simulink model "FullFMS_2026_02_25_V0_4_31_R2026a"  (R2026a)
settings: Solver=FixedStepAuto  StopTime=inf  FixedStep=0.01  MaxStep=0.01  RelTol=1e-2
PreLoadFcn:
  | load("BUS_CONFIG.mat")
libraries: opcualib x8
(part 3 of 4)

== stateflow chart FullFMS_2026_02_25_V0_4_31_R2026a/Chart ==
  note: Conveyor
  note: Sorting [60]
  state BRS
    entry:
    StatusBRS_5 = false;   % v0.4.29: zera o fim de ciclo anterior
    state STATE1
      entry:
      StatusBRS_1 = false;
      during:
      % Configuracao da estacao: so este bloco fica ativo se o bit dele estiver ligado
      if Control_60.C_65_BRS_Output
      StatusBRS_1 = true;
      else
      StatusBRS_1 = false;
      end
    state ESTATE2
      entry:
      StatusBRS_2 = false;
      during:
      % Janela de identificacao da peca (T1 = 2s no ladder)
      if Control_50.C_55_PD_Sort
      StatusBRS_2 = true;
      else
      StatusBRS_2 = false;
      end
    state ESTATE3
      entry:
      StatusBRS_3 = false;
      during:
      % Preta: SL1 avanca | Vermelha: SL2 avanca | Prata: ambas recuadas
      if ((Control_60.C_65_ID_1 && ~Control_60.C_65_ID_2) && Sensors_60.O_60_SL1_Fwd) || ...
      ((Control_60.C_65_ID_1 && Control_60.C_65_ID_2) && Sensors_60.O_60_SL2_Fwd) || ...
      ((~Control_60.C_65_ID_1 && Control_60.C_65_ID_2) && Sensors_60.O_60_SL1_Bck && Sensors_60.O_60_SL2_Bck)
      StatusBRS_3 = true;
      else
      StatusBRS_3 = false;
      end
    state ESTATE5
      entry:
      StatusBRS_5 = false;
      during:
      % Pino recuado: ciclo concluido, pronto para a proxima peca
      if ~Actuators_60.F_62_Identify
      StatusBRS_5 = true;
      else
      StatusBRS_5 = false;
      end
    state ESTATE4
      entry:
      % captura no mesmo passo da entrada
      StatusBRS_4 = Actuators_60.F_62_Identify;
      during:
      % Pino de identificacao acionado (LEITURA do CLP - sombra nao comanda)
      % latch (v0.4.31): o pino desliga junto com o Part_Pass, uma vez observado nao volta a false
      if Actuators_60.F_62_Identify
      StatusBRS_4 = true;
      end
    (default) -> BRS.STATE1
    BRS.ESTATE2 -> BRS.ESTATE3 : [(Control_60.C_65_ID_1 == true || Control_60.C_65_ID_2 == true || after(2, sec)) && StatusBRS_2 == true]
    BRS.ESTATE3 -> BRS.ESTATE4 : [StatusBRS_3 == true]
    BRS.ESTATE4 -> BRS.ESTATE5 : [(Sensors_60.O_60_Part_Pass == true || Actuators_60.F_62_Identify == false) && StatusBRS_4 == true]
    BRS.STATE1 -> BRS.ESTATE2 : [Control_50.C_55_PD_Sort == true && StatusBRS_1 == true]
  state Start
    during:
    Control_20.C_24_Request
  note: Testing Station [70]
  note: Distribution Station [80]
  state Identified_Delivery
    state Part_HeightSensor
      entry:
      St_IdDl_3a_8 = false;
      during:
      Actuators_70.F_72_Eject_Part;
      Sensors_70.O_70_Pist_Bck;
      Sensors_70.O_70_SPart_Height
      if Actuators_70.F_72_Eject_Part && ...
      ~Sensors_70.O_70_Pist_Bck && ...
      ~Sensors_70.O_70_SPart_Height
      St_IdDl_3a_8 = true;
      else
      St_IdDl_3a_8 = false;
      end
    state Piston_Back
      entry:
      Status3a_10 = false;
      during:
      Actuators_70.F_72_Eject_Part
      if ~Actuators_70.F_72_Eject_Part
      Status3a_10 = true;
      else
      Status3a_10 = false;
      end
    state Elevator_StartsMovingDown
      entry:
      Status3a_11 = false;
      during:
      Actuators_70.F_72_Elev_Down;
      Actuators_70.F_72_Elev_Up;
      if Actuators_70.F_72_Elev_Down && ...
      ~Actuators_70.F_72_Elev_Up
      Status3a_11 = true;
      else
      Status3a_11 = false;
      end
    state Elevator_MiddleDown
      entry:
      Status3a_12 = false;
      during:
      Sensors_70.O_70_SStation;
      if ~Sensors_70.O_70_SStation
      Status3a_12 = true;
      else
      Status3a_12 = false;
      end
    state Elevator_InductiveDown
      entry:
      St_IdDl_3a_13 = false;
      during:
      Sensors_70.O_70_SInductive;
      if ~Sensors_70.O_70_SInductive
      St_IdDl_3a_13 = true;
      else
      St_IdDl_3a_13 = false;
      end
    state Pushes_Part
      entry:
      Status3a_7 = false;
      during:
      Actuators_70.F_72_Eject_Part;
      Actuators_70.F_72_Air_On;
      Sensors_70.O_70_SPart;
      if Actuators_70.F_72_Eject_Part && ...
      Actuators_70.F_72_Air_On && ...
      ~Sensors_70.O_70_SPart
      Status3a_7 = true;
      else
      Status3a_7 = false;
      end
    state InitialCondition
      entry:
      St_IdDl_3a_1 = false;
      during:
      AS_i_70.A_74_Cart_Full;
      Control_70.C_75_Initialization;
      Control_70.C_72_Profibus;
      Control_70.C_75_Identified;
      Sensors_70.O_70_SPart;
      Sensors_70.O_71_Key_Pos;
      if ~AS_i_70.A_74_Cart_Full && ...
      Control_70.C_75_Initialization && ...
      Control_70.C_72_Profibus && ...
      Control_70.C_75_Identified && ...
      ~Sensors_70.O_70_SPart && ...
      Sensors_70.O_71_Key_Pos
      St_IdDl_3a_1 = true;
      else
      St_IdDl_3a_1 = false;
      end
    state Part_Arrives
      entry:
      Status3a_2 = false;
      during:
      Control_70.C_75_ID_Delivery2;
      Sensors_70.O_70_SInductive;
      Sensors_70.O_70_SPart;
      Sensors_80.O_80_Arm_Mag;
      if Sensors_70.O_70_SPart && ...
      ((Sensors_70.O_70_SInductive && ...
      Control_70.C_75_ID_Delivery2) | ...
      (~Sensors_70.O_70_SInductive && ...
      ~Control_70.C_75_ID_Delivery2)) && ...
      ~Sensors_80.O_80_Arm_Mag
      Status3a_2 = true;
      else
      Status3a_2 =false;
      end
    state Elevator_Up
      entry:
      Status3a_3 = false;
      during:
      Actuators_70.F_72_Elev_Up;
      if Actuators_70.F_72_Elev_Up
      Status3a_3 = true;
      else
      Status3a_3 = false;
      end
    state Elevator_StartsMovingUp
      entry:
      Status3a_4 = false;
      during:
      Sensors_70.O_70_SInductive;
      if ~Sensors_70.O_70_SInductive
      Status3a_4 = true;
      else
      Status3a_4 = false;
      end
    state Elevator_MiddleUp
      entry:
      Status3a_5 = false;
      during:
      Sensors_70.O_70_SStation;
      if ~Sensors_70.O_70_SStation
      Status3a_5 = true;
      else
      Status3a_5 = false;
      end
    state Elevator_High_Identify_Part
      entry:
      Status3a_6 = false;
      during:
      MetalicPart;
      Control_70.C_75_ID_Delivery1;
      Control_70.C_75_ID_Delivery2;
      Sensors_70.O_70_SPart_Height;
      if MetalicPart && ...
      Control_70.C_75_ID_Delivery2 && ...
      ~Control_70.C_75_ID_Delivery1;
      Status3a_6 = true;
      end
      if ~MetalicPart && ...
      Control_70.C_75_ID_Delivery1 && ...
      ((Sensors_70.O_70_SPart_Height && ...
      Control_70.C_75_ID_Delivery2) | ...
      (~Sensors_70.O_70_SPart_Height && ...
      ~Control_70.C_75_ID_Delivery2))
      Status3a_6=true;
      end
    state Elevator_Down
      entry:
      Status3a_14 = false;
      during:
      AS_i_70.A_74_CRoute_Out;
      Actuators_70.F_72_Elev_Down;
      Control_70.C_75_Part_Del;
      if AS_i_70.A_74_CRoute_Out && ...
      ~Actuators_70.F_72_Elev_Down&& ...
      Control_70.C_75_Part_Del
      Status3a_14 = true;
      else
      Status3a_14 = false;
      end
    state Part_ArrivesAtCart
      entry:
      Status3a_9 = false;
      during:
      AS_i_70.A_74_Cart_Full;
      AS_i_70.A_74_Optic;
      Actuators_70.F_72_Air_On;
      Actuators_70.F_73_Led_Extra2
      if AS_i_70.A_74_Optic && ...
      AS_i_70.A_74_Cart_Full && ...
      ~Actuators_70.F_72_Air_On && ...
      Actuators_70.F_73_Led_Extra2;
      Status3a_9 = true;
      else
      Status3a_9 = false;
      end
    state End_Process
      entry:
      Status3a_15 = false;
      during:
      AS_i_70.A_74_CRoute_Out;
      if  ~AS_i_70.A_74_CRoute_Out
      Status3a_15 = true;
      else
      Status3a_15 = false;
      end
    state Metalic_Identify
      entry:
      MetalicPart = false;
      during:
      Sensors_70.O_70_SInductive;
      if Sensors_70.O_70_SInductive
      MetalicPart = true;
      else
      MetalicPart = false;
      end
    (default) -> Identified_Delivery.InitialCondition
    Identified_Delivery.Elevator_StartsMovingDown -> Identified_Delivery.Elevator_MiddleDown : [Status3a_11 == true && ...
        | Sensors_70.O_70_SStation == true]
    Identified_Delivery.Piston_Back -> Identified_Delivery.Elevator_StartsMovingDown : [Status3a_10 == true && ...
        | Sensors_70.O_70_Pist_Bck == true]
    Identified_Delivery.Elevator_MiddleDown -> Identified_Delivery.Elevator_InductiveDown : [Status3a_12 == true && ...
        | Sensors_70.O_70_SInductive == true]
    Identified_Delivery.Part_Arrives -> Identified_Delivery.Elevator_Up : [Status3a_2 == true && ...
        | Sensors_80.O_80_Arm_Mag == true ]
    Identified_Delivery.Elevator_High_Identify_Part -> Identified_Delivery.Pushes_Part : [Status3a_6 == true && ...
        | (Actuators_70.F_72_Eject_Part == true || after(2, sec))]
    Identified_Delivery.Pushes_Part -> Identified_Delivery.Part_HeightSensor : [Status3a_7 == true && ...
        | Sensors_70.O_70_Pist_Bck == false]
    Identified_Delivery.Elevator_Up -> Identified_Delivery.Elevator_StartsMovingUp : [Status3a_3 == true && ...
        | Sensors_70.O_70_SInductive == true ]
    Identified_Delivery.Elevator_InductiveDown -> Identified_Delivery.Elevator_Down : [St_IdDl_3a_13 == true && ...
        | Sensors_70.O_70_Elev_Low == true]
    Identified_Delivery.Part_HeightSensor -> (junction 1354)
    (junction 1354) -> Identified_Delivery.Piston_Back [order 1] : [St_IdDl_3a_8 == true && ...
        | (Sensors_70.O_70_Pist_Bck == true || after(2, sec))]
    Identified_Delivery.Elevator_StartsMovingUp -> Identified_Delivery.Elevator_MiddleUp : [Status3a_4 == true && ...
        | Sensors_70.O_70_SStation == true]
    Identified_Delivery.Elevator_MiddleUp -> Identified_Delivery.Elevator_High_Identify_Part : [Status3a_5 == true && ...
        | Sensors_70.O_70_Elev_High == true]
    Identified_Delivery.InitialCondition -> (junction 1348) : [St_IdDl_3a_1 == true && ...
        | Sensors_70.O_70_SPart == true]
    (junction 1348) -> Identified_Delivery.Part_Arrives [order 1]
    (junction 1354) -> (junction 1356) [order 2] : [St_IdDl_3a_8 == true && ...
        | AS_i_70.A_74_Optic == true]
    (junction 1348) -> (junction 1350) [order 2]
    Identified_Delivery.Elevator_Down -> Identified_Delivery.End_Process : [Sensors_70.O_70_Elev_Low == true && Control_70.C_75_Part_Del == true]
    (junction 1356) -> Identified_Delivery.Part_ArrivesAtCart
    (junction 1350) -> Identified_Delivery.Metalic_Identify
  state Distribution_Single
    state PistonStartsMoveBackward
      entry:
      St_DSg0_2a_7 = false;
      during:
      Sensors_80.O_80_Pist_Fwd;
      if ~Sensors_80.O_80_Pist_Fwd
      St_DSg0_2a_7 = true;
      else
      St_DSg0_2a_7 = false;
      end
    state PartFed
      entry:
      St_DSg0_2a_6 = false;
      during:
      Actuators_80.F_82_Pist_Adv;
      if ~Actuators_80.F_82_Pist_Adv
      St_DSg0_2a_6 = true;
      else
      St_DSg0_2a_6 = false;
      end
    state ArmToMagazine
      entry:
      St_DSg0_2a_8 = false;
      during:
      Actuators_80.F_82_Arm_2_Mag;
      if Actuators_80.F_82_Arm_2_Mag
      St_DSg0_2a_8 = true;
      else
      St_DSg0_2a_8 = false;
      end
    state ArmCloseDeliver1
      entry:
      St_DSg0_2a_9 = false;
      during:
      Sensors_70.O_70_SStation;
      if Sensors_70.O_70_SStation
      St_DSg0_2a_9 = true;
      else
      St_DSg0_2a_9 = false;
      end
    state ArmArrives_PicksPart
      entry:
      St_DSg0_2a_10 = false;
      during:
      Actuators_80.F_82_Suction_On;
      Actuators_80.F_82_Arm_2_Mag;
      if Actuators_80.F_82_Suction_On && ...
      ~Actuators_80.F_82_Arm_2_Mag
      St_DSg0_2a_10 = true;
      else
      St_DSg0_2a_10 = false;
      end
    state ArmToDelivery1
      entry:
      St_DSg0_2a_11 = false;
      during:
      Actuators_80.F_82_Arm_2_Del
      if Actuators_80.F_82_Arm_2_Del
      St_DSg0_2a_11 = true;
      else
      St_DSg0_2a_11 = false;
      end
    state ArmCloseDelivery2
      entry:
      St_DSg0_2a_12 = false;
      during:
      Sensors_70.O_70_SStation;
      if Sensors_70.O_70_SStation
      St_DSg0_2a_12 = true;
      else
      St_DSg0_2a_12 = false;
      end
    state ArmArrives_DeliversPart
      entry:
      St_DSg0_2a_13 = false;
      during:
      Actuators_80.F_82_Suction_On;
      Actuators_80.F_82_Suction_Off;
      Actuators_80.F_82_Arm_2_Del;
      if ~Actuators_80.F_82_Suction_On && ...
      Actuators_80.F_82_Suction_Off && ...
      ~Actuators_80.F_82_Arm_2_Del
      St_DSg0_2a_13 = true;
      else
      St_DSg0_2a_13 = false;
      end
    state ArmToMagazine1
      entry:
      St_DSg0_2a_14 = false;
      during:
      Actuators_80.F_82_Suction_Off;
      Actuators_80.F_82_Arm_2_Mag;
      Actuators_80.F_83_Led_Extra1;
      Control_80.C_85_Part_Del;
      if ~Actuators_80.F_82_Suction_Off && ...
      Actuators_80.F_82_Arm_2_Mag && ...
      Actuators_80.F_83_Led_Extra1 && ...
      Control_80.C_85_Part_Del
      St_DSg0_2a_14 = true;
      else
      St_DSg0_2a_14 = false;
      end
    state ArmCloseDeliver3
      entry:
      St_DSg0_2a_15 = false;
      during:
      Sensors_70.O_70_SStation;
      if Sensors_70.O_70_SStation
      St_DSg0_2a_15 = true;
      else
      St_DSg0_2a_15 = false;
      end
    state ArmArrives_Finish
      entry:
      St_DSg0_2a_16 = false;
      during:
      Actuators_80.F_82_Arm_2_Mag;
      if ~Actuators_80.F_82_Arm_2_Mag
      St_DSg0_2a_16 = true;
      else
      St_DSg0_2a_16 = false;
      end
    state InitialCondition
      entry:
      St_DSg0_2a_1 = false;
      during:
      Control_80.C_85_Initialization;
      Control_80.C_86_Mag_Parts;
      Control_80.C_82_Profibus;
      Control_80.C_85_Single;
      Sensors_80.O_80_Arm_Mag;
      Sensors_80.O_81_Key_Pos;
      if Control_80.C_85_Initialization&& ...
      Control_80.C_86_Mag_Parts ~= 0 && ...
      Control_80.C_82_Profibus && ...
      Control_80.C_85_Single && ...
      Sensors_80.O_80_Arm_Mag && ...
      Sensors_80.O_81_Key_Pos
      St_DSg0_2a_1 = true;
      else
      St_DSg0_2a_1 = false;
      end
    state ArmToDelivery
      entry:
      St_DSg0_2a_2 = false;
      during:
      Actuators_80.F_82_Arm_2_Del;
      if Actuators_80.F_82_Arm_2_Del
      St_DSg0_2a_2 = true;
      else
      St_DSg0_2a_2 = false;
      end
    state ArmCloseDelivery
      entry:
      St_DSg0_2a_3 = false;
      during:
      Sensors_70.O_70_SStation;
      if Sensors_70.O_70_SStation
      St_DSg0_2a_3 = true;
      else
      St_DSg0_2a_3 = false;
      end
    state ArmArrives_FeedsPart
      entry:
      St_DSg0_2a_4 = false;
      during:
      Actuators_80.F_82_Pist_Adv;
      Actuators_80.F_82_Arm_2_Del;
      if Actuators_80.F_82_Pist_Adv && ...
      ~Actuators_80.F_82_Arm_2_Del
      St_DSg0_2a_4 = true;
      else
      St_DSg0_2a_4 = false;
      end
    state PistonStartsMoveForward
      entry:
      St_DSg0_2a_5 = false;
      during:
      Sensors_80.O_80_Pist_Bck;
      if ~Sensors_80.O_80_Pist_Bck
      St_DSg0_2a_5 = true;
      else
      St_DSg0_2a_5 = false;
      end
    state T1
      during:
      Control_80.C_85_Part_Del
      Actuators_80.F_83_Led_Extra1
    (default) -> Distribution_Single.InitialCondition
    Distribution_Single.ArmToMagazine1 -> (junction 650)
    (junction 650) -> Distribution_Single.ArmCloseDeliver3 [order 1] : [Sensors_80.O_80_Arm_Del == false &&...
        |  St_DSg0_2a_14 == true]
    Distribution_Single.ArmToDelivery -> Distribution_Single.ArmCloseDelivery : [Sensors_80.O_80_Arm_Mag == false &&...
        |  St_DSg0_2a_2 == true]
    Distribution_Single.ArmCloseDelivery -> Distribution_Single.ArmArrives_FeedsPart : [Sensors_80.O_80_Arm_Del == true && ...
        | St_DSg0_2a_3 == true]
    Distribution_Single.ArmArrives_DeliversPart -> Distribution_Single.ArmToMagazine1 : [Sensors_80.O_80_Part_Stuck == false && ...
        | St_DSg0_2a_13 == true]
    Distribution_Single.ArmCloseDelivery2 -> Distribution_Single.ArmArrives_DeliversPart : [Sensors_80.O_80_Arm_Del == true && ...
        | St_DSg0_2a_12 == true]
    Distribution_Single.ArmArrives_FeedsPart -> Distribution_Single.PistonStartsMoveForward : [St_DSg0_2a_4 == true]
    Distribution_Single.PistonStartsMoveBackward -> Distribution_Single.ArmToMagazine : [Sensors_80.O_80_Pist_Bck == true && ...
        | St_DSg0_2a_7 == true]
    Distribution_Single.ArmCloseDeliver1 -> Distribution_Single.ArmArrives_PicksPart : [Sensors_80.O_80_Arm_Mag == true && ...
        | St_DSg0_2a_9 == true]
    Distribution_Single.PartFed -> Distribution_Single.PistonStartsMoveBackward : [St_DSg0_2a_6 == true]
    Distribution_Single.ArmToMagazine -> Distribution_Single.ArmCloseDeliver1 : [Sensors_80.O_80_Arm_Del == false &&...
        | St_DSg0_2a_8 == true]
    Distribution_Single.InitialCondition -> Distribution_Single.ArmToDelivery : [Sensors_80.O_81_Start == true | ...
        | Control_80.C_85_Start == true | ...
        | Control_70.C_75_RQ_Wrong == true | ...
        | (AS_i_70.A_74_CRoute_In80 == true && Sensors_80.O_81_Key_Pos == true) ]
    Distribution_Single.ArmCloseDeliver3 -> Distribution_Single.ArmArrives_Finish : [Sensors_80.O_80_Arm_Mag == true && ...
        | St_DSg0_2a_15 == true]
    Distribution_Single.ArmToDelivery1 -> Distribution_Single.ArmCloseDelivery2 : [Sensors_80.O_80_Arm_Mag == false &&...
        | St_DSg0_2a_11 == true]
    Distribution_Single.PistonStartsMoveForward -> Distribution_Single.PartFed : [Sensors_80.O_80_Pist_Fwd == true && ...
        | St_DSg0_2a_5 == true]
    Distribution_Single.ArmArrives_PicksPart -> Distribution_Single.ArmToDelivery1 : [Sensors_80.O_80_Part_Stuck == true && ...
        | St_DSg0_2a_10 == true]
    (junction 650) -> (junction 1222) [order 2] : after(4,sec)
    (junction 1222) -> Distribution_Single.T1
  state BSR
    entry:
    StatusBSR_5 = false;   % v0.4.29: zera o fim de ciclo anterior
    state STATE1
      entry:
      StatusBSR_1 = false;
      during:
      % Configuracao da estacao: so este bloco fica ativo se o bit dele estiver ligado
      if Control_60.C_65_BSR_Output
      StatusBSR_1 = true;
      else
      StatusBSR_1 = false;
      end
    state ESTATE2
      entry:
      StatusBSR_2 = false;
      during:
      % Janela de identificacao da peca (T1 = 2s no ladder)
      if Control_50.C_55_PD_Sort
      StatusBSR_2 = true;
      else
      StatusBSR_2 = false;
      end
    state ESTATE3
      entry:
      StatusBSR_3 = false;
      during:
      % Preta: SL1 avanca | Prata: SL2 avanca | Vermelha: ambas recuadas
      if ((Control_60.C_65_ID_1 && ~Control_60.C_65_ID_2) && Sensors_60.O_60_SL1_Fwd) || ...
      ((~Control_60.C_65_ID_1 && Control_60.C_65_ID_2) && Sensors_60.O_60_SL2_Fwd) || ...
      ((Control_60.C_65_ID_1 && Control_60.C_65_ID_2) && Sensors_60.O_60_SL1_Bck && Sensors_60.O_60_SL2_Bck)
      StatusBSR_3 = true;
      else
      StatusBSR_3 = false;
      end
    state ESTATE4
      entry:
      % captura no mesmo passo da entrada
      StatusBSR_4 = Actuators_60.F_62_Identify;
      during:
      % Pino de identificacao acionado (LEITURA do CLP - sombra nao comanda)
      % latch (v0.4.31): o pino desliga junto com o Part_Pass, uma vez observado nao volta a false
      if Actuators_60.F_62_Identify
      StatusBSR_4 = true;
      end
    state ESTATE5
      entry:
      StatusBSR_5 = false;
      during:
      % Pino recuado: ciclo concluido, pronto para a proxima peca
      if ~Actuators_60.F_62_Identify
      StatusBSR_5 = true;
      else
      StatusBSR_5 = false;
      end
    (default) -> BSR.STATE1
    BSR.ESTATE3 -> BSR.ESTATE4 : [StatusBSR_3 == true]
    BSR.ESTATE2 -> BSR.ESTATE3 : [(Control_60.C_65_ID_1 == true || Control_60.C_65_ID_2 == true || after(2, sec)) && StatusBSR_2 == true]
    BSR.STATE1 -> BSR.ESTATE2 : [Control_50.C_55_PD_Sort == true && StatusBSR_1 == true]
    BSR.ESTATE4 -> BSR.ESTATE5 : [(Sensors_60.O_60_Part_Pass == true || Actuators_60.F_62_Identify == false) && StatusBSR_4 == true]
  note: Handling 1 [50]
  state Distribution_Continuous
    state InitialCondition
      entry:
      St_DCt0_2b_1 = false;
      during:
      Control_80.C_85_Initialization;
      Control_80.C_86_Mag_Parts;
      Control_80.C_82_Profibus;
      Control_80.C_85_Continuous;
      Sensors_80.O_80_Arm_Mag;
      Sensors_80.O_81_Key_Pos;
      if Control_80.C_85_Initialization&& ...
      Control_80.C_86_Mag_Parts ~= 0 && ...
      Control_80.C_82_Profibus && ...
      Control_80.C_85_Continuous && ...
      Sensors_80.O_80_Arm_Mag && ...
      Sensors_80.O_81_Key_Pos
      St_DCt0_2b_1 = true;
      else
      St_DCt0_2b_1 = false;
      end
    state ArmToDelivery
      entry:
      St_DCt0_2b_2 = false;
      during:
      Actuators_80.F_82_Arm_2_Del
      if Actuators_80.F_82_Arm_2_Del
      St_DCt0_2b_2 = true;
      else
      St_DCt0_2b_2 = false;
      end
    state ArmCloseDelivery
      entry:
      St_DCt0_2b_3 = false;
      during:
      Sensors_70.O_70_SStation;
      if Sensors_70.O_70_SStation
      St_DCt0_2b_3 = true;
      else
      St_DCt0_2b_3 = false;
      end
    state ArmArrives_FeedsPart
      entry:
      St_DCt0_2b_4 = false;
      during:
      Actuators_80.F_82_Pist_Adv;
      Actuators_80.F_82_Arm_2_Del;
      if Actuators_80.F_82_Pist_Adv && ...
      ~Actuators_80.F_82_Arm_2_Del
      St_DCt0_2b_4 = true;
      else
      St_DCt0_2b_4 = false;
      end
    state PistonStartsMoveForward
      entry:
      St_DCt0_2b_5 = false;
      during:
      Sensors_80.O_80_Pist_Bck;
      if ~Sensors_80.O_80_Pist_Bck
      St_DCt0_2b_5 = true;
      else
      St_DCt0_2b_5 = false;
      end
    state PartFed
      entry:
      St_DCt0_2b_6 = false;
      during:
      Actuators_80.F_82_Pist_Adv;
      if ~Actuators_80.F_82_Pist_Adv
      St_DCt0_2b_6 = true;
      else
      St_DCt0_2b_6 = false;
      end
    state PistonStartsMoveBackward
      entry:
      St_DCt0_2b_7 = false;
      during:
      Sensors_80.O_80_Pist_Fwd;
      if ~Sensors_80.O_80_Pist_Fwd
      St_DCt0_2b_7 = true;
      else
      St_DCt0_2b_7 = false;
      end
    state ArmToMagazine
      entry:
      St_DCt0_2b_8 = false;
      during:
      Actuators_80.F_82_Arm_2_Mag;
      if Actuators_80.F_82_Arm_2_Mag
      St_DCt0_2b_8 = true;
      else
      St_DCt0_2b_8 = false;
      end
    state ArmCloseDeliver1
      entry:
      St_DCt0_2b_9 = false;
      during:
      Sensors_70.O_70_SStation;
      if Sensors_70.O_70_SStation
      St_DCt0_2b_9 = true;
      else
      St_DCt0_2b_9 = false;
      end
    state ArmArrives_PicksPart
      entry:
      St_DCt0_2b_10 = false;
      during:
      Actuators_80.F_82_Suction_On;
      Actuators_80.F_82_Arm_2_Mag;
      if Actuators_80.F_82_Suction_On && ...
      ~Actuators_80.F_82_Arm_2_Mag
      St_DCt0_2b_10 = true;
      else
      St_DCt0_2b_10 = false;
      end
    state ArmToDelivery1
      entry:
      St_DCt0_2b_11 = false;
      during:
      Actuators_80.F_82_Arm_2_Del
      if Actuators_80.F_82_Arm_2_Del
      St_DCt0_2b_11 = true;
      else
      St_DCt0_2b_11 = false;
      end
    state ArmCloseDelivery2
      entry:
      St_DCt0_2b_12 = false;
      during:
      Sensors_70.O_70_SStation;
      if Sensors_70.O_70_SStation
      St_DCt0_2b_12 = true;
      else
      St_DCt0_2b_12 = false;
      end
    state ArmArrives_DeliversPart
      entry:
      St_DCt0_2b_13 = false;
      during:
      Actuators_80.F_82_Suction_On;
      Actuators_80.F_82_Suction_Off;
      Actuators_80.F_82_Arm_2_Del;
      if ~Actuators_80.F_82_Suction_On && ...
      Actuators_80.F_82_Suction_Off && ...
      ~Actuators_80.F_82_Arm_2_Del
      St_DCt0_2b_13 = true;
      else
      St_DCt0_2b_13 = false;
      end
    state PartDel_CheckLoop
      entry:
      LoopDistCont = false;
      during:
      Control_80.C_85_Part_Del
      Sensors_80.O_80_Mag_Empty
      if Control_80.C_85_Part_Del && ...
      ~Sensors_80.O_80_Mag_Empty
      LoopDistCont = true;
      else
      LoopDistCont = false;
      end
    state ArmToMagazine1
      entry:
      St_DCt0_2b_14 = false;
      during:
      Actuators_80.F_82_Suction_Off;
      Actuators_80.F_82_Arm_2_Mag;
      Actuators_80.F_83_Led_Extra1;
      Control_80.C_85_Part_Del;
      if ~Actuators_80.F_82_Suction_Off && ...
      Actuators_80.F_82_Arm_2_Mag && ...
      Actuators_80.F_83_Led_Extra1 && ...
      Control_80.C_85_Part_Del
      St_DCt0_2b_14 = true;
      else
      St_DCt0_2b_14 = false;
      end
    state ArmCloseDeliver3
      entry:
      St_DCt0_2b_15 = false;
      during:
      Sensors_70.O_70_SStation;
      if Sensors_70.O_70_SStation
      St_DCt0_2b_15 = true;
      else
      St_DCt0_2b_15 = false;
      end
    state ArmArrives_Finish
      entry:
      St_DCt0_2b_16 = false;
      during:
      Actuators_80.F_82_Arm_2_Mag;
      if ~Actuators_80.F_82_Arm_2_Mag
      St_DCt0_2b_16 = true;
      else
      St_DCt0_2b_16 = false;
      end
    state T1
      during:
      Control_80.C_85_Part_Del
      Actuators_80.F_83_Led_Extra1
    Distribution_Continuous.ArmArrives_PicksPart -> Distribution_Continuous.ArmToDelivery1 : [Sensors_80.O_80_Part_Stuck == true && ...
        | St_DCt0_2b_10 == true]
    Distribution_Continuous.ArmArrives_DeliversPart -> Distribution_Continuous.PartDel_CheckLoop : [Sensors_80.O_80_Part_Stuck == false && ...
        | St_DCt0_2b_13 == true]
    Distribution_Continuous.ArmCloseDelivery -> Distribution_Continuous.ArmArrives_FeedsPart : [Sensors_80.O_80_Arm_Del == true && ...
        | St_DCt0_2b_3 == true]
    Distribution_Continuous.ArmArrives_FeedsPart -> Distribution_Continuous.PistonStartsMoveForward : [St_DCt0_2b_4 == true]
    (default) -> Distribution_Continuous.InitialCondition
    Distribution_Continuous.PartFed -> Distribution_Continuous.PistonStartsMoveBackward : [St_DCt0_2b_6 == true]
    Distribution_Continuous.PistonStartsMoveForward -> Distribution_Continuous.PartFed : [Sensors_80.O_80_Pist_Fwd == true && ...
        | St_DCt0_2b_5 == true]
    Distribution_Continuous.ArmToDelivery -> Distribution_Continuous.ArmCloseDelivery : [Sensors_80.O_80_Arm_Mag == false &&...
        | St_DCt0_2b_2 == true]
    Distribution_Continuous.PistonStartsMoveBackward -> Distribution_Continuous.ArmToMagazine : [Sensors_80.O_80_Pist_Bck == true && ...
        | St_DCt0_2b_7 == true]
    Distribution_Continuous.ArmCloseDelivery2 -> Distribution_Continuous.ArmArrives_DeliversPart : [Sensors_80.O_80_Arm_Del == true && ...
        | St_DCt0_2b_12 == true]
    Distribution_Continuous.ArmToMagazine -> Distribution_Continuous.ArmCloseDeliver1 : [Sensors_80.O_80_Arm_Del == false &&...
        |  St_DCt0_2b_8 == true]
    Distribution_Continuous.ArmCloseDeliver1 -> Distribution_Continuous.ArmArrives_PicksPart : [Sensors_80.O_80_Arm_Mag == true && ...
        | St_DCt0_2b_9 == true]
    Distribution_Continuous.ArmToDelivery1 -> Distribution_Continuous.ArmCloseDelivery2 : [Sensors_80.O_80_Arm_Mag == false &&...
        |  St_DCt0_2b_11 == true]
    Distribution_Continuous.InitialCondition -> Distribution_Continuous.ArmToDelivery : [Sensors_80.O_81_Start == true | ...
        | Control_80.C_85_Start == true | ...
        | (AS_i_70.A_74_CRoute_In80 == true && Sensors_80.O_81_Key_Pos == true) ]
    Distribution_Continuous.ArmToMagazine1 -> Distribution_Continuous.ArmCloseDeliver3 : [Sensors_80.O_80_Arm_Del == false &&...
        | St_DCt0_2b_14 == true]
    Distribution_Continuous.ArmCloseDeliver3 -> Distribution_Continuous.ArmArrives_Finish : [Sensors_80.O_80_Arm_Mag == true && ...
        | St_DCt0_2b_15 == true]
    Distribution_Continuous.PartDel_CheckLoop -> Distribution_Continuous.ArmToMagazine1 [order 2] : [LoopDistCont == false]
    (junction 708) -> Distribution_Continuous.ArmArrives_FeedsPart
    (junction 706) -> (junction 708)
    Distribution_Continuous.PartDel_CheckLoop -> (junction 707) [order 1] : [LoopDistCont == true]
    Distribution_Continuous.PartDel_CheckLoop -> Distribution_Continuous.T1 [order 3] : after(4,sec)
    (junction 707) -> (junction 706)
  state Handling1_Cart2Del
    state Config_H1
      entry:
      St_H1_1 = false;
      during:
      % FB4 Cart_2_Del - entrega do Conveyor para a Sorting
      if Control_50.C_55_Initialization
      St_H1_1 = true;
      else
      St_H1_1 = false;
      end
    state Aguarda_H1
      entry:
      St_H1_2 = false;
      during:
      % N1: condicoes para iniciar o transporte
      if (Sensors_50.O_51_Start || Control_50.C_55_Start || (AS_i_50.A_54_CRoute_In && Sensors_50.O_51_Key_Pos)) && ...
      AS_i_50.A_54_Cart_Stat && AS_i_50.A_54_Optic && ~Sensors_60.O_60_SPart
      St_H1_2 = true;
      else
      St_H1_2 = false;
      end
    state DesceVazia_H1
      entry:
      St_H1_3 = false;
      during:
      % N2: desce a garra vazia sobre o carro
      if ~Control_50.C_55_PD_Sort && Sensors_50.O_50_Claw_Cart && Sensors_50.O_50_Claw_High && ~Sensors_50.O_50_Part_in_Claw && Actuators_50.F_52_Claw_Down
      St_H1_3 = true;
      else
      St_H1_3 = false;
      end
    state PegaPeca_H1
      entry:
      St_H1_4 = false;
      during:
      % N3: fecha a garra e levanta com a peca
      if Sensors_50.O_50_Claw_Cart && Sensors_50.O_50_Claw_Low && Actuators_50.F_52_Close_Claw
      St_H1_4 = true;
      else
      St_H1_4 = false;
      end
    state MoveEntrega_H1
      entry:
      St_H1_5 = false;
      during:
      % N4: move a garra ate a posicao de entrega
      if Sensors_50.O_50_Claw_High && Sensors_50.O_50_Part_in_Claw && ~Sensors_50.O_50_Claw_Del && Actuators_50.F_52_Claw_2_Del
      St_H1_5 = true;
      else
      St_H1_5 = false;
      end
    state DesceEntrega_H1
      entry:
      St_H1_6 = false;
      during:
      % N5: desce a garra para entregar
      if Sensors_50.O_50_Claw_Del && Sensors_50.O_50_Claw_High && Sensors_50.O_50_Part_in_Claw && Actuators_50.F_52_Claw_Down
      St_H1_6 = true;
      else
      St_H1_6 = false;
      end
    state EntregaPeca_H1
      entry:
      St_H1_7 = false;
      during:
      % N6: abre a garra e solta a peca
      if Sensors_50.O_50_Claw_Del && Sensors_50.O_50_Claw_Low && ~Actuators_50.F_52_Close_Claw
      St_H1_7 = true;
      else
      St_H1_7 = false;
      end
    state SinalizaEntrega_H1
      entry:
      St_H1_8 = false;
      during:
      % N7: sinaliza peca entregue na Sorting
      if Sensors_50.O_50_Claw_Del && Sensors_50.O_50_Claw_High && ~Sensors_50.O_50_Part_in_Claw && Control_50.C_55_PD_Sort
      St_H1_8 = true;
      else
      St_H1_8 = false;
      end
    state VoltaGarra_H1
      entry:
      St_H1_9 = false;
      during:
      % N8/N9: volta a garra ao carro e prepara sinal de roteamento
      if Control_50.C_55_PD_Sort && Actuators_50.F_52_Claw_2_Cart && (Sensors_50.O_50_Claw_Cart || AS_i_50.A_54_CRoute_Out)
      St_H1_9 = true;
      else
      St_H1_9 = false;
      end
    (default) -> Config_H1
    Config_H1 -> Aguarda_H1 : [St_H1_1 == true]
    Aguarda_H1 -> DesceVazia_H1 : [St_H1_2 == true]
    DesceVazia_H1 -> PegaPeca_H1 : [St_H1_3 == true]
    PegaPeca_H1 -> MoveEntrega_H1 : [St_H1_4 == true]
    MoveEntrega_H1 -> DesceEntrega_H1 : [St_H1_5 == true]
    DesceEntrega_H1 -> EntregaPeca_H1 : [St_H1_6 == true]
    EntregaPeca_H1 -> SinalizaEntrega_H1 : [St_H1_7 == true]
    SinalizaEntrega_H1 -> VoltaGarra_H1 : [St_H1_8 == true]
  state Requested_Delivery
    state Part_HeightSensor
      entry:
      Status3b_8 = false;
      during:
      Actuators_70.F_72_Eject_Part;
      Sensors_70.O_70_Pist_Bck;
      Sensors_70.O_70_SPart_Height
      if Actuators_70.F_72_Eject_Part && ...
      ~Sensors_70.O_70_Pist_Bck && ...
      ~Sensors_70.O_70_SPart_Height
      Status3b_8 = true;
      else
      Status3b_8 = false;
      end
    state Piston_Back
      entry:
      Status3b_10 = false;
      during:
      Actuators_70.F_72_Eject_Part
      if ~Actuators_70.F_72_Eject_Part
      Status3b_10 = true;
      else
      Status3b_10 = false;
      end
    state Elevator_StartsMovingDown
      entry:
      Status3b_11 = false;
      during:
      Actuators_70.F_72_Elev_Down;
      Actuators_70.F_72_Elev_Up;
      if Actuators_70.F_72_Elev_Down && ...
      ~Actuators_70.F_72_Elev_Up
      Status3b_11 = true;
      else
      Status3b_11 = false;
      end
    state Elevator_MiddleDown
      entry:
      Status3b_12 = false;
      during:
      Sensors_70.O_70_SStation;
      if ~Sensors_70.O_70_SStation
      Status3b_12 = true;
      else
      Status3b_12 = false;
      end
    state Elevator_InductiveDown
      entry:
      Status3b_13 = false;
      during:
      Sensors_70.O_70_SInductive;
      if ~Sensors_70.O_70_SInductive
      Status3b_13 = true;
      else
      Status3b_13 = false;
      end
    state InitialCondition
      entry:
      Status3b_1 = false;
      during:
      AS_i_70.A_74_Cart_Full;
      Control_70.C_75_Initialization;
      Control_70.C_72_Profibus;
      Control_70.C_75_Requested;
      Sensors_70.O_70_SPart;
      Sensors_70.O_71_Key_Pos;
      if ~AS_i_70.A_74_Cart_Full && ...
      Control_70.C_75_Initialization && ...
      Control_70.C_72_Profibus && ...
      Control_70.C_75_Requested && ...
      ~Sensors_70.O_70_SPart && ...
      Sensors_70.O_71_Key_Pos
      Status3b_1 = true;
      else
      Status3b_1 = false;
      end
    state Part_Arrives
      entry:
      Status3b_2 = false;
      during:
      Control_70.C_75_ID_Delivery2;
      Sensors_70.O_70_SInductive;
      Sensors_70.O_70_SPart;
      Sensors_80.O_80_Arm_Mag;
      if Sensors_70.O_70_SPart && ...
      ((Sensors_70.O_70_SInductive && ...
      Control_70.C_75_ID_Delivery2) | ...
      (~Sensors_70.O_70_SInductive && ...
      ~Control_70.C_75_ID_Delivery2)) && ...
      ~Sensors_80.O_80_Arm_Mag
      Status3b_2 = true;
      else
      Status3b_2 =false;
      end
    state Elevator_Up
      entry:
      Status3b_3 = false;
      during:
      Actuators_70.F_72_Elev_Up;
      if Actuators_70.F_72_Elev_Up
      Status3b_3 = true;
      else
      Status3b_3 = false;
      end
    state Elevator_StartsMovingUp
      entry:
      Status3b_4 = false;
      during:
      Sensors_70.O_70_SInductive;
      if ~Sensors_70.O_70_SInductive
      Status3b_4 = true;
      else
      Status3b_4 = false;
      end
    state Elevator_MiddleUp
      entry:
      Status3b_5 = false;
      during:
      Sensors_70.O_70_SStation;
      if ~Sensors_70.O_70_SStation
      Status3b_5 = true;
      else
      Status3b_5 = false;
      end
    state Elevator_High_Identify_Part
      entry:
      Status3b_6 = false;
      during:
      MetalicPart;
      Control_70.C_75_ID_Delivery1;
      Control_70.C_75_ID_Delivery2;
      Sensors_70.O_70_SPart_Height;
      if MetalicPart && ...
      Control_70.C_75_ID_Delivery2 && ...
      ~Control_70.C_75_ID_Delivery1;
      Status3b_6 = true;
      end
      if ~MetalicPart && ...
      Control_70.C_75_ID_Delivery1 && ...
      ((Sensors_70.O_70_SPart_Height && ...
      Control_70.C_75_ID_Delivery2) | ...
      (~Sensors_70.O_70_SPart_Height && ...
      ~Control_70.C_75_ID_Delivery2))
      Status3b_6=true;
      end
    state CheckPart
      entry:
      Part_Equal = false;
      Part_Different = false;
      during:
      Control_70.C_75_ID_Delivery1;
      Control_70.C_75_ID_Delivery2;
      Control_70.C_75_RQ_Delivery1;
      Control_70.C_75_RQ_Delivery2;
      if (Control_70.C_75_ID_Delivery1 == ...
      Control_70.C_75_RQ_Delivery1) && ...
      (Control_70.C_75_ID_Delivery2 == ...
      Control_70.C_75_RQ_Delivery2)
      Part_Equal = true;
      else
      Part_Different = true;
      end
    state Pushes_Part
      entry:
      Status3b_7 = false;
      during:
      Actuators_70.F_72_Eject_Part;
      Actuators_70.F_72_Air_On;
      Sensors_70.O_70_SPart;
      if Actuators_70.F_72_Eject_Part && ...
      Actuators_70.F_72_Air_On && ...
      ~Sensors_70.O_70_SPart
      Status3b_7 = true;
      else
      Status3b_7 = false;
      end
    state Elevator_Down
      entry:
      Status3b_14 = false;
      during:
      AS_i_70.A_74_CRoute_Out;
      Actuators_70.F_72_Elev_Down;
      Control_70.C_75_Part_Del;
      if AS_i_70.A_74_CRoute_Out && ...
      ~Actuators_70.F_72_Elev_Down&& ...
      Control_70.C_75_Part_Del
      Status3b_14 = true;
      else
      Status3b_14 = false;
      end
    state Part_ArrivesAtCart
      entry:
      Status3b_9 = false;
      during:
      AS_i_70.A_74_Cart_Full;
      AS_i_70.A_74_Optic;
      Actuators_70.F_72_Air_On;
      Actuators_70.F_73_Led_Extra2
      if AS_i_70.A_74_Optic && ...
      AS_i_70.A_74_Cart_Full && ...
      ~Actuators_70.F_72_Air_On && ...
      Actuators_70.F_73_Led_Extra2;
      Status3b_9 = true;
      else
      Status3b_9 = false;
      end
    state End_Process
      entry:
      Status3b15 = false;
      during:
      AS_i_70.A_74_CRoute_Out;
      if  ~AS_i_70.A_74_CRoute_Out
      Status3b_15 = true;
      else
      Status3b_15 = false;
      end
    state Metalic_Identify
      entry:
      MetalicPart = false;
      during:
      Sensors_70.O_70_SInductive;
      if Sensors_70.O_70_SInductive
      MetalicPart = true;
      else
      MetalicPart = false;
      end
    state Elevator_StartsMovingDown1
      entry:
      Status3b_16 = false;
      during:
      Actuators_70.F_72_Elev_Down;
      Actuators_70.F_72_Elev_Up;
      if Actuators_70.F_72_Elev_Down && ...
      ~Actuators_70.F_72_Elev_Up
      Status3b_16 = true;
      else
      Status3b_16 = false;
      end
    state Elevator_MiddleDown1
      entry:
      Status3b_17 = false;
      during:
      Sensors_70.O_70_SStation;
      if ~Sensors_70.O_70_SStation
      Status3b_17 = true;
      else
      Status3b_17 = false;
      end
    state Elevator_InductiveDown1
      entry:
      Status3b_18 = false;
      during:
      Sensors_70.O_70_SInductive;
      if ~Sensors_70.O_70_SInductive
      Status3b_18 = true;
      else
      Status3b_18 = false;
      end
    state Elevator_Down1
      entry:
      Status3b_19 = false;
      during:
      Actuators_70.F_72_Eject_Part
      Actuators_70.F_72_Elev_Down
      if Actuators_70.F_72_Eject_Part && ...
      ~Actuators_70.F_72_Elev_Down
      Status3b_19 = true;
      else
      Status3b_19 = false;
      end
    state Piston_Back1
      entry:
      Status3b_20 = false;
      during:
      Actuators_70.F_72_Eject_Part
      Sensors_70.O_70_Pist_Bck;
      Sensors_70.O_70_SPart
      Control_70.C_75_RQ_Wrong;
      if ~Actuators_70.F_72_Eject_Part && ...
      Sensors_70.O_70_Pist_Bck && ...
      ~Sensors_70.O_70_SPart && ...
      Control_70.C_75_RQ_Wrong;
      Status3b_20 = true;
      else
      Status3b_20 = false;
      end
    (default) -> Requested_Delivery.InitialCondition
    Requested_Delivery.Elevator_StartsMovingDown -> Requested_Delivery.Elevator_MiddleDown : [Status3b_11 == true && ...
        | Sensors_70.O_70_SStation == true]
    Requested_Delivery.Piston_Back -> Requested_Delivery.Elevator_StartsMovingDown : [Status3b_10 == true && ...
        | Sensors_70.O_70_Pist_Bck == true]
    Requested_Delivery.Elevator_MiddleDown -> Requested_Delivery.Elevator_InductiveDown : [Status3b_12 == true && ...
        | Sensors_70.O_70_SInductive == true]
    Requested_Delivery.Part_Arrives -> Requested_Delivery.Elevator_Up : [Status3b_2 == true && ...
        | Sensors_80.O_80_Arm_Mag == true ]
    Requested_Delivery.Pushes_Part -> Requested_Delivery.Part_HeightSensor : [Status3b_7 == true && ...
        | Sensors_70.O_70_Pist_Bck == false]
    Requested_Delivery.Elevator_Up -> Requested_Delivery.Elevator_StartsMovingUp : [Status3b_3 == true && ...
        | Sensors_70.O_70_SInductive == true ]
    Requested_Delivery.Elevator_StartsMovingUp -> Requested_Delivery.Elevator_MiddleUp : [Status3b_4 == true && ...
        | Sensors_70.O_70_SStation == true]
    Requested_Delivery.Elevator_MiddleUp -> Requested_Delivery.Elevator_High_Identify_Part : [Status3b_5 == true && ...
        | Sensors_70.O_70_Elev_High == true]
    Requested_Delivery.Elevator_InductiveDown -> Requested_Delivery.Elevator_Down : [Status3b_13 == true && ...
        | Sensors_70.O_70_Elev_Low == true]
    Requested_Delivery.Part_HeightSensor -> (junction 1412)
    (junction 1412) -> Requested_Delivery.Piston_Back [order 1] : [Status3b_8 == true && ...
        | (Sensors_70.O_70_Pist_Bck == true || after(2, sec))]
    Requested_Delivery.Elevator_High_Identify_Part -> CheckPart : [Status3b_6 == true && ...
        | (Actuators_70.F_72_Eject_Part == true || after(2, sec))]
    CheckPart -> (junction 1378)
    (junction 1378) -> Requested_Delivery.Pushes_Part [order 1] : [Part_Equal == true]
    Requested_Delivery.InitialCondition -> (junction 1372) : [Status3b_1 == true && ...
        | Sensors_70.O_70_SPart == true]
    (junction 1372) -> Requested_Delivery.Part_Arrives [order 1]
    (junction 1412) -> (junction 1410) [order 2] : [Status3b_8 == true && ...
        | AS_i_70.A_74_Optic == true]
    (junction 1378) -> (junction 952) [order 2] : [Part_Different == true]
    (junction 1372) -> (junction 1376) [order 2]
    Requested_Delivery.Elevator_Down -> Requested_Delivery.End_Process : [Sensors_70.O_70_Elev_Low == true && Control_70.C_75_Part_Del == true]
    (junction 1410) -> Requested_Delivery.Part_ArrivesAtCart
    (junction 1376) -> Requested_Delivery.Metalic_Identify
    Elevator_MiddleDown1 -> Elevator_InductiveDown1 : [Status3b_17 == true && ...
        | Sensors_70.O_70_SInductive == true]
    Elevator_StartsMovingDown1 -> Elevator_MiddleDown1 : [Status3b_16 == true && ...
        | Sensors_70.O_70_SStation == true]
    Elevator_Down1 -> Piston_Back1 : [Status3b_19 == true && ...
        | Sensors_70.O_70_Pist_Bck == false]
    (junction 952) -> Elevator_StartsMovingDown1
    Elevator_InductiveDown1 -> Elevator_Down1 : [Status3b_18 == true && ...
        | Sensors_70.O_70_Elev_Low == true]
  state Distribution_Counted
    state ArmToMagazine1
      entry:
      St_DCd0_2c_14 = false;
      during:
      Actuators_80.F_82_Suction_Off;
      Actuators_80.F_82_Arm_2_Mag;
      Actuators_80.F_83_Led_Extra1;
      Control_80.C_85_Part_Del;
      if ~Actuators_80.F_82_Suction_Off && ...
      Actuators_80.F_82_Arm_2_Mag && ...
      Actuators_80.F_83_Led_Extra1 && ...
      Control_80.C_85_Part_Del
      St_DCd0_2c_14 = true;
      else
      St_DCd0_2c_14 = false;
      end
    state ArmCloseDeliver3
      entry:
      St_DCd0_2c_15 = false;
      during:
      Sensors_70.O_70_SStation;
      if Sensors_70.O_70_SStation
      St_DCd0_2c_15 = true;
      else
      St_DCd0_2c_15 = false;
      end
    state ArmArrives_Finish
      entry:
      St_DCd0_2c_16 = false;
      during:
      Actuators_80.F_82_Arm_2_Mag;
      if ~Actuators_80.F_82_Arm_2_Mag
      St_DCd0_2c_16 = true;
      else
      St_DCd0_2c_16 = false;
      end
    state ArmToMagazine
      entry:
      St_DCd0_2c_8 = false;
      during:
      Actuators_80.F_82_Arm_2_Mag;
      if Actuators_80.F_82_Arm_2_Mag
      St_DCd0_2c_8 = true;
      else
      St_DCd0_2c_8 = false;
      end
    state ArmCloseDeliver1
      entry:
      St_DCd0_2c_9 = false;
      during:
      Sensors_70.O_70_SStation;
      if Sensors_70.O_70_SStation
      St_DCd0_2c_9 = true;
      else
      St_DCd0_2c_9 = false;
      end
    state ArmArrives_PicksPart
      entry:
      St_DCd0_2c_10 = false;
      during:
      Actuators_80.F_82_Suction_On;
      Actuators_80.F_82_Arm_2_Mag;
      if Actuators_80.F_82_Suction_On && ...
      ~Actuators_80.F_82_Arm_2_Mag
      St_DCd0_2c_10 = true;
      else
      St_DCd0_2c_10 = false;
      end
    state ArmToDelivery1
      entry:
      St_DCd0_2c_11 = false;
      during:
      Actuators_80.F_82_Arm_2_Del
      if Actuators_80.F_82_Arm_2_Del
      St_DCd0_2c_11 = true;
      else
      St_DCd0_2c_11 = false;
      end
    state ArmCloseDelivery2
      entry:
      St_DCd0_2c_12 = false;
      during:
      Sensors_70.O_70_SStation;
      if Sensors_70.O_70_SStation
      St_DCd0_2c_12 = true;
      else
      St_DCd0_2c_12 = false;
      end
    state ArmArrives_DeliversPart
      entry:
      St_DCd0_2c_13 = false;
      during:
      Actuators_80.F_82_Suction_On;
      Actuators_80.F_82_Suction_Off;
      Actuators_80.F_82_Arm_2_Del;
      if ~Actuators_80.F_82_Suction_On && ...
      Actuators_80.F_82_Suction_Off && ...
      ~Actuators_80.F_82_Arm_2_Del
      St_DCd0_2c_13 = true;
      else
      St_DCd0_2c_13 = false;
      end
    state PartDel_CheckLoop
      entry:
      LoopDistCont = false;
      during:
      Control_80.C_85_Part_Del
      Control_80.C_87_RQ_MParts
      if Control_80.C_85_Part_Del && ...
      Control_80.C_87_RQ_MParts ~= 0
      LoopDistCont = true;
      else
      LoopDistCont = false;
      end
    state InitialCondition
      entry:
      St_DCd0_2c_1 = false;
      during:
      Control_80.C_85_Initialization;
      Control_80.C_86_Mag_Parts;
      Control_80.C_83_RQ_Parts;
      Control_80.C_82_Profibus;
      Control_80.C_85_Counted;
      Sensors_80.O_80_Arm_Mag;
      Sensors_80.O_81_Key_Pos;
      if Control_80.C_85_Initialization&& ...
      Control_80.C_86_Mag_Parts ~= 0 && ...
      Control_80.C_86_Mag_Parts >= Control_80.C_83_RQ_Parts && ...
      Control_80.C_82_Profibus && ...
      Control_80.C_85_Counted && ...
      Sensors_80.O_80_Arm_Mag && ...
      Sensors_80.O_81_Key_Pos
      St_DCd0_2c_1 = true;
      else
      St_DCd0_2c_1 = false;
      end
    state ArmToDelivery
      entry:
      St_DCd0_2c_2 = false;
      during:
      Actuators_80.F_82_Arm_2_Del
      if Actuators_80.F_82_Arm_2_Del
      St_DCd0_2c_2 = true;
      else
      St_DCd0_2c_2 = false;
      end
    state ArmCloseDelivery
      entry:
      St_DCd0_2c_3 = false;
      during:
      Sensors_70.O_70_SStation;
      if Sensors_70.O_70_SStation
      St_DCd0_2c_3 = true;
      else
      St_DCd0_2c_3 = false;
      end
    state ArmArrives_FeedsPart
      entry:
      St_DCd0_2c_4 = false;
      during:
      Actuators_80.F_82_Pist_Adv;
      Actuators_80.F_82_Arm_2_Del;
      if Actuators_80.F_82_Pist_Adv && ...
      ~Actuators_80.F_82_Arm_2_Del
      St_DCd0_2c_4 = true;
      else
      St_DCd0_2c_4 = false;
      end
    state PistonStartsMoveForward
      entry:
      St_DCd0_2c_5 = false;
      during:
      Sensors_80.O_80_Pist_Bck;
      if ~Sensors_80.O_80_Pist_Bck
      St_DCd0_2c_5 = true;
      else
      St_DCd0_2c_5 = false;
      end
    state PartFed
      entry:
      St_DCd0_2c_6 = false;
      during:
      Actuators_80.F_82_Pist_Adv;
      if ~Actuators_80.F_82_Pist_Adv
      St_DCd0_2c_6 = true;
      else
      St_DCd0_2c_6 = false;
      end
    state PistonStartsMoveBackward
      entry:
      St_DCd0_2c_7 = false;
      during:
      Sensors_80.O_80_Pist_Fwd;
      if ~Sensors_80.O_80_Pist_Fwd
      St_DCd0_2c_7 = true;
      else
      St_DCd0_2c_7 = false;
      end
    state T1
      during:
      Control_80.C_85_Part_Del
      Actuators_80.F_83_Led_Extra1
    Distribution_Counted.InitialCondition -> Distribution_Counted.ArmToDelivery : [Sensors_80.O_81_Start == true | ...
        | Control_80.C_85_Start == true | ...
        | (AS_i_70.A_74_CRoute_In80 == true && Sensors_80.O_81_Key_Pos == true) ]
    Distribution_Counted.ArmArrives_FeedsPart -> Distribution_Counted.PistonStartsMoveForward : [St_DCd0_2c_4 == true]
    Distribution_Counted.PartDel_CheckLoop -> Distribution_Counted.ArmToMagazine1 [order 2] : [LoopDistCont == false]
    Distribution_Counted.ArmCloseDeliver3 -> Distribution_Counted.ArmArrives_Finish : [Sensors_80.O_80_Arm_Mag == true && ...
        | St_DCd0_2c_15 == true]
    Distribution_Counted.ArmCloseDelivery2 -> Distribution_Counted.ArmArrives_DeliversPart : [Sensors_80.O_80_Arm_Del == true && ...
        | St_DCd0_2c_12 == true]
    Distribution_Counted.ArmCloseDelivery -> Distribution_Counted.ArmArrives_FeedsPart : [Sensors_80.O_80_Arm_Del == true && ...
        | St_DCd0_2c_3 == true]
    Distribution_Counted.PistonStartsMoveForward -> Distribution_Counted.PartFed : [Sensors_80.O_80_Pist_Fwd == true && ...
        | St_DCd0_2c_5 == true]
    Distribution_Counted.ArmArrives_DeliversPart -> Distribution_Counted.PartDel_CheckLoop : [Sensors_80.O_80_Part_Stuck == false && ...
        | St_DCd0_2c_13 == true]
    Distribution_Counted.ArmToMagazine1 -> Distribution_Counted.ArmCloseDeliver3 : [Sensors_80.O_80_Arm_Del == false &&...
        | St_DCd0_2c_14 == true]
    Distribution_Counted.ArmArrives_PicksPart -> Distribution_Counted.ArmToDelivery1 : [Sensors_80.O_80_Part_Stuck == true && ...
        | St_DCd0_2c_10 == true]
    Distribution_Counted.PistonStartsMoveBackward -> Distribution_Counted.ArmToMagazine : [Sensors_80.O_80_Pist_Bck == true && ...
        | St_DCd0_2c_7 == true]
    Distribution_Counted.ArmToDelivery -> Distribution_Counted.ArmCloseDelivery : [Sensors_80.O_80_Arm_Mag == false &&...
        | St_DCd0_2c_2 == true]
    Distribution_Counted.ArmToMagazine -> Distribution_Counted.ArmCloseDeliver1 : [Sensors_80.O_80_Arm_Del == false &&...
        | St_DCd0_2c_8 == true]
    Distribution_Counted.ArmCloseDeliver1 -> Distribution_Counted.ArmArrives_PicksPart : [Sensors_80.O_80_Arm_Mag == true && ...
        | St_DCd0_2c_9 == true]
    Distribution_Counted.PartFed -> Distribution_Counted.PistonStartsMoveBackward : [St_DCd0_2c_6 == true]
    (default) -> Distribution_Counted.InitialCondition
    Distribution_Counted.ArmToDelivery1 -> Distribution_Counted.ArmCloseDelivery2 : [Sensors_80.O_80_Arm_Mag == false &&...
        | St_DCd0_2c_11 == true]
    (junction 804) -> Distribution_Counted.ArmArrives_FeedsPart
    (junction 820) -> (junction 804)
    Distribution_Counted.PartDel_CheckLoop -> (junction 821) [order 1] : [LoopDistCont == true]
    Distribution_Counted.PartDel_CheckLoop -> Distribution_Counted.T1 [order 3] : after(4,sec)
    (junction 821) -> (junction 820)
  state RBS
    entry:
    StatusRBS_5 = false;   % v0.4.29: zera o fim de ciclo anterior
    state STATE2
      entry:
      StatusRBS_1 = false;
      during:
      % Configuracao da estacao: so este bloco fica ativo se o bit dele estiver ligado
      if Control_60.C_65_RBS_Output
      StatusRBS_1 = true;
      else
      StatusRBS_1 = false;
      end
    state ESTATE7
      entry:
      StatusRBS_2 = false;
      during:
      % Janela de identificacao da peca (T1 = 2s no ladder)
      if Control_50.C_55_PD_Sort
      StatusRBS_2 = true;
      else
      StatusRBS_2 = false;
      end
    state ESTATE9
      entry:
      StatusRBS_3 = false;
      during:
      % Vermelha: SL1 avanca | Preta: SL2 avanca | Prata: ambas recuadas
      if ((Control_60.C_65_ID_1 && Control_60.C_65_ID_2) && Sensors_60.O_60_SL1_Fwd) || ...
      ((Control_60.C_65_ID_1 && ~Control_60.C_65_ID_2) && Sensors_60.O_60_SL2_Fwd) || ...
      ((~Control_60.C_65_ID_1 && Control_60.C_65_ID_2) && Sensors_60.O_60_SL1_Bck && Sensors_60.O_60_SL2_Bck)
      StatusRBS_3 = true;
      else
      StatusRBS_3 = false;
      end
    state ESTATE6
      entry:
      % captura no mesmo passo da entrada
      StatusRBS_4 = Actuators_60.F_62_Identify;
      during:
      % Pino de identificacao acionado (LEITURA do CLP - sombra nao comanda)
      % latch (v0.4.31): o pino desliga junto com o Part_Pass, uma vez observado nao volta a false
      if Actuators_60.F_62_Identify
      StatusRBS_4 = true;
      end
    state ESTATE8
      entry:
      StatusRBS_5 = false;
      during:
      % Pino recuado: ciclo concluido, pronto para a proxima peca
      if ~Actuators_60.F_62_Identify
      StatusRBS_5 = true;
      else
      StatusRBS_5 = false;
      end
    (default) -> STATE2
    ESTATE9 -> ESTATE6 : [StatusRBS_3 == true]
    STATE2 -> ESTATE7 : [Control_50.C_55_PD_Sort == true && StatusRBS_1 == true]
    ESTATE7 -> ESTATE9 : [(Control_60.C_65_ID_1 == true || Control_60.C_65_ID_2 == true || after(2, sec)) && StatusRBS_2 == true]
    ESTATE6 -> ESTATE8 : [(Sensors_60.O_60_Part_Pass == true || Actuators_60.F_62_Identify == false) && StatusRBS_4 == true]
  note: Conveyor
  note: Processing [100]
  note: Conveyor
  state RSB
    entry:
    StatusRSB_5 = false;   % v0.4.29: zera o fim de ciclo anterior
    state STATE1
      entry:
      StatusRSB_1 = false;
      during:
      % Configuracao da estacao: so este bloco fica ativo se o bit dele estiver ligado
      if Control_60.C_65_RSB_Output
      StatusRSB_1 = true;
      else
      StatusRSB_1 = false;
      end
    state ESTATE2
      entry:
      StatusRSB_2 = false;
      during:
      % Janela de identificacao da peca (T1 = 2s no ladder)
      if Control_50.C_55_PD_Sort
      StatusRSB_2 = true;
      else
      StatusRSB_2 = false;
      end
    state ESTATE3
      entry:
      StatusRSB_3 = false;
      during:
      % Vermelha: SL1 avanca | Prata: SL2 avanca | Preta: ambas recuadas
      if ((Control_60.C_65_ID_1 && Control_60.C_65_ID_2) && Sensors_60.O_60_SL1_Fwd) || ...
      ((~Control_60.C_65_ID_1 && Control_60.C_65_ID_2) && Sensors_60.O_60_SL2_Fwd) || ...
      ((Control_60.C_65_ID_1 && ~Control_60.C_65_ID_2) && Sensors_60.O_60_SL1_Bck && Sensors_60.O_60_SL2_Bck)
      StatusRSB_3 = true;
      else
      StatusRSB_3 = false;
      end
    state ESTATE4
      entry:
      % captura no mesmo passo da entrada
      StatusRSB_4 = Actuators_60.F_62_Identify;
      during:
      % Pino de identificacao acionado (LEITURA do CLP - sombra nao comanda)
      % latch (v0.4.31): o pino desliga junto com o Part_Pass, uma vez observado nao volta a false
      if Actuators_60.F_62_Identify
      StatusRSB_4 = true;
      end
    state ESTATE5
      entry:
      StatusRSB_5 = false;
      during:
      % Pino recuado: ciclo concluido, pronto para a proxima peca
      if ~Actuators_60.F_62_Identify
      StatusRSB_5 = true;
      else
      StatusRSB_5 = false;
      end
    (default) -> RSB.STATE1
    RSB.ESTATE4 -> RSB.ESTATE5 : [(Sensors_60.O_60_Part_Pass == true || Actuators_60.F_62_Identify == false) && StatusRSB_4 == true]
    RSB.ESTATE3 -> RSB.ESTATE4 : [StatusRSB_3 == true]
    RSB.ESTATE2 -> RSB.ESTATE3 : [(Control_60.C_65_ID_1 == true || Control_60.C_65_ID_2 == true || after(2, sec)) && StatusRSB_2 == true]
    RSB.STATE1 -> RSB.ESTATE2 : [Control_50.C_55_PD_Sort == true && StatusRSB_1 == true]
  note: Handling 2 [90]
  note: Storage [40]
  state Processing_TestOnly
    state GiraTeste_TOnly
      entry:
      St_TOnly_3 = false;
      during:
      % N2: mesa girando ate a posicao de teste (contador C4, preset 4)
      if Actuators_100.F_102_RT_On
      St_TOnly_3 = true;
      else
      St_TOnly_3 = false;
      end
    state Config_TOnly
      entry:
      St_TOnly_1 = false;
      during:
      % FB4 Test Part Only - bloco ativo so neste modo
      if Control_100.C_105_Test && ~Control_100.C_105_TestDrill && ~Control_100.C_105_Rotation
      St_TOnly_1 = true;
      else
      St_TOnly_1 = false;
      end
    state Aguarda_TOnly
      entry:
      St_TOnly_2 = false;
      during:
      % N1: condicoes para iniciar o ciclo de teste
      if Sensors_100.O_100_PInit_Pos && Sensors_90.O_90_Claw_High && Sensors_100.O_100_RT_Sensor && ~Actuators_100.F_102_RT_On
      St_TOnly_2 = true;
      else
      St_TOnly_2 = false;
      end
    state PosTeste_TOnly
      entry:
      St_TOnly_4 = false;
      during:
      % N3: peca na posicao de teste, temporizador de 2s
      if ~Actuators_100.F_102_RT_On && Sensors_100.O_100_PTest_Pos && Sensors_100.O_100_RT_Sensor
      St_TOnly_4 = true;
      else
      St_TOnly_4 = false;
      end
    state Testando_TOnly
      entry:
      St_TOnly_5 = false;
      during:
      % N4: pino de teste acionado
      if Actuators_100.F_102_Test_Pin
      St_TOnly_5 = true;
      else
      St_TOnly_5 = false;
      end
    state Resultado_TOnly
      entry:
      St_TOnly_6 = false;
      during:
      % N5/N6: PTest_Ok define OK ou Falha (Profibus)
      if Control_100.C_105_Test_Ok || Control_100.C_105_Test_Fail
      St_TOnly_6 = true;
      else
      St_TOnly_6 = false;
      end
    state Retirada_TOnly
      entry:
      St_TOnly_7 = false;
      during:
      % N1(R): peca retirada pela garra da HD2, reseta o ciclo
      if Sensors_90.O_90_Claw_Del && Sensors_90.O_90_Claw_Low && Sensors_90.O_90_Part_in_Claw
      St_TOnly_7 = true;
      else
      St_TOnly_7 = false;
      end
    (default) -> Config_TOnly
    Resultado_TOnly -> Retirada_TOnly : [St_TOnly_6 == true]
    GiraTeste_TOnly -> PosTeste_TOnly : [St_TOnly_3 == true]
    PosTeste_TOnly -> Testando_TOnly : [St_TOnly_4 == true && (Actuators_100.F_102_Test_Pin == true || after(2, sec))]
    Testando_TOnly -> Resultado_TOnly : [St_TOnly_5 == true]
    Aguarda_TOnly -> GiraTeste_TOnly : [St_TOnly_2 == true]
    Config_TOnly -> Aguarda_TOnly : [St_TOnly_1 == true]
  state PartToProcessing
    state Config_P2P0
      entry:
      % captura no mesmo passo da entrada
      St_P2P0_5_1 = Control_90.C_95_Initialization && Control_90.C_92_Profibus && Control_90.C_95_Cart2Del;
      during:
      % OB1 N5 / FB4 N1: inicia o transporte carro --> entrega
      % latch, como as bobinas S do FB: uma vez observado, nao volta a false
      if Control_90.C_95_Initialization && Control_90.C_92_Profibus && Control_90.C_95_Cart2Del
      St_P2P0_5_1 = true;
      end
    state GarraNoCarro_P2P0
      entry:
      % captura no mesmo passo da entrada
      St_P2P0_5_2 = Actuators_90.F_92_Claw_2_Cart || Sensors_90.O_90_Claw_Cart;
      during:
      % FB4 N2: garante a garra na posicao do carro
      % latch, como as bobinas S do FB: uma vez observado, nao volta a false
      if Actuators_90.F_92_Claw_2_Cart || Sensors_90.O_90_Claw_Cart
      St_P2P0_5_2 = true;
      end
    state DescePega_P2P0
      entry:
      % captura no mesmo passo da entrada
      St_P2P0_5_3 = ( Sensors_90.O_90_Claw_Cart && Actuators_90.F_92_Claw_Down && Sensors_90.O_90_Claw_Low ) || ...
      ( Sensors_90.O_90_Claw_Cart && Sensors_90.O_90_Part_in_Claw );
      during:
      % FB4: desce a garra no carro (ou: ja esta com a peca no carro -> a descida ocorreu)
      % latch, como as bobinas S do FB: uma vez observado, nao volta a false
      if ( Sensors_90.O_90_Claw_Cart && Actuators_90.F_92_Claw_Down && Sensors_90.O_90_Claw_Low ) || ...
      ( Sensors_90.O_90_Claw_Cart && Sensors_90.O_90_Part_in_Claw )
      St_P2P0_5_3 = true;
      end
    state FechaGarra_P2P0
      entry:
      % captura no mesmo passo da entrada
      St_P2P0_5_4 = Actuators_90.F_92_Close_Claw && Sensors_90.O_90_Part_in_Claw;
      during:
      % FB4 N3: fecha a garra e pega a peca
      % latch, como as bobinas S do FB: uma vez observado, nao volta a false
      if Actuators_90.F_92_Close_Claw && Sensors_90.O_90_Part_in_Claw
      St_P2P0_5_4 = true;
      end
    state SobeComPeca_P2P0
      entry:
      % captura no mesmo passo da entrada
      St_P2P0_5_5 = Sensors_90.O_90_Part_in_Claw && Sensors_90.O_90_Claw_High && ~Actuators_90.F_92_Claw_Down;
      during:
      % FB4 N4: sobe com a peca
      % latch, como as bobinas S do FB: uma vez observado, nao volta a false
      if Sensors_90.O_90_Part_in_Claw && Sensors_90.O_90_Claw_High && ~Actuators_90.F_92_Claw_Down
      St_P2P0_5_5 = true;
      end
    state MoveParaEntrega_P2P0
      entry:
      % captura no mesmo passo da entrada
      St_P2P0_5_6 = Sensors_90.O_90_Claw_Del && Sensors_90.O_90_Part_in_Claw;
      during:
      % FB4: braco chegou a entrega com a peca (F_92_Claw_2_Del cai ao chegar, por isso nao entra)
      % latch, como as bobinas S do FB: uma vez observado, nao volta a false
      if Sensors_90.O_90_Claw_Del && Sensors_90.O_90_Part_in_Claw
      St_P2P0_5_6 = true;
      end
    state DesceEntrega_P2P0
      entry:
      % captura no mesmo passo da entrada
      St_P2P0_5_7 = ( Sensors_90.O_90_Claw_Del && Actuators_90.F_92_Claw_Down && Sensors_90.O_90_Claw_Low ) || ...
      ( Sensors_90.O_90_Claw_Del && ~Sensors_90.O_90_Part_in_Claw );
      during:
      % FB4: desce na entrega (ou: ja soltou a peca na entrega -> a descida ocorreu)
      % latch, como as bobinas S do FB: uma vez observado, nao volta a false
      if ( Sensors_90.O_90_Claw_Del && Actuators_90.F_92_Claw_Down && Sensors_90.O_90_Claw_Low ) || ...
      ( Sensors_90.O_90_Claw_Del && ~Sensors_90.O_90_Part_in_Claw )
      St_P2P0_5_7 = true;
      end
    state AbreGarra_P2P0
      entry:
      % captura no mesmo passo da entrada
      St_P2P0_5_8 = ~Actuators_90.F_92_Close_Claw && ~Sensors_90.O_90_Part_in_Claw;
      during:
      % FB4 N5: abre a garra e solta a peca
      % latch, como as bobinas S do FB: uma vez observado, nao volta a false
      if ~Actuators_90.F_92_Close_Claw && ~Sensors_90.O_90_Part_in_Claw
      St_P2P0_5_8 = true;
      end
    state SobeVazia_P2P0
      entry:
      % captura no mesmo passo da entrada
      St_P2P0_5_9 = Sensors_90.O_90_Claw_High && ~Sensors_90.O_90_Part_in_Claw;
      during:
      % FB4 N6: sobe sem a peca
      % latch, como as bobinas S do FB: uma vez observado, nao volta a false
      if Sensors_90.O_90_Claw_High && ~Sensors_90.O_90_Part_in_Claw
      St_P2P0_5_9 = true;
      end
    state PecaEntregue_P2P0
      entry:
      % captura no mesmo passo da entrada
      St_P2P0_5_10 = Control_90.C_95_PD_Proc;
      during:
      % FB4 N6: sinaliza peca entregue na Processing
      % latch, como as bobinas S do FB: uma vez observado, nao volta a false
      if Control_90.C_95_PD_Proc
      St_P2P0_5_10 = true;
      end
    (default) -> Config_P2P0
    Config_P2P0 -> GarraNoCarro_P2P0 : [St_P2P0_5_1 == true]
    GarraNoCarro_P2P0 -> DescePega_P2P0 : [St_P2P0_5_2 == true]
    DescePega_P2P0 -> FechaGarra_P2P0 : [St_P2P0_5_3 == true]
    FechaGarra_P2P0 -> SobeComPeca_P2P0 : [St_P2P0_5_4 == true]
    SobeComPeca_P2P0 -> MoveParaEntrega_P2P0 : [St_P2P0_5_5 == true]
    MoveParaEntrega_P2P0 -> DesceEntrega_P2P0 : [St_P2P0_5_6 == true]
    DesceEntrega_P2P0 -> AbreGarra_P2P0 : [St_P2P0_5_7 == true]
    AbreGarra_P2P0 -> SobeVazia_P2P0 : [St_P2P0_5_8 == true]
    SobeVazia_P2P0 -> PecaEntregue_P2P0 : [St_P2P0_5_9 == true]
  state Store
    state Config_Stor
      entry:
      St_Stor_1 = false;
      during:
      % FB4 Store Part - bloco ativo so no modo armazenar
      if Control_40.C_45_Initialization && Control_40.C_45_StorePart
      St_Stor_1 = true;
      else
      St_Stor_1 = false;
      end
    state Aguarda_Stor
      entry:
      St_Stor_2 = false;
      during:
      % OB1 N4: carro chegou e comando de armazenar presente
      if (Control_40.C_45_Start || (AS_i_40.A_44_CRoute_In && Sensors_40.O_41_Key_Pos)) && AS_i_40.A_44_Cart_Stat
      St_Stor_2 = true;
      else
      St_Stor_2 = false;
      end
    state Armazenando_Stor
      entry:
      St_Stor_3 = false;
      during:
      % FB4 N1: temporizador simulado T1 = 3s (S5T#3S)
      % A estacao nao tem mecanica real: o CLP so conta o tempo.
      if Control_40.C_45_StorePart
      St_Stor_3 = true;
      else
      St_Stor_3 = false;
      end
    state ProcessoOK_Stor
      entry:
      St_Stor_4 = false;
      during:
      % OB1 N6: fim do procedimento, sinaliza processo concluido
      if Control_40.C_45_StorePart
      St_Stor_4 = true;
      else
      St_Stor_4 = false;
      end
    state LiberaCarro_Stor
      entry:
      St_Stor_5 = false;
      during:
      % OB1 N7: pulso de 2s libera o carro (A_44_CRoute_Out)
      if AS_i_40.A_44_CRoute_Out || ~AS_i_40.A_44_Cart_Stat
      St_Stor_5 = true;
      else
      St_Stor_5 = false;
      end
    (default) -> Config_Stor
    Config_Stor -> Aguarda_Stor : [St_Stor_1 == true]
    Aguarda_Stor -> Armazenando_Stor : [St_Stor_2 == true]
    Armazenando_Stor -> ProcessoOK_Stor : [St_Stor_3 == true && after(3, sec)]
    ProcessoOK_Stor -> LiberaCarro_Stor : [St_Stor_4 == true]
  state Processing_TestDrill
    state Retirada_TDrill
      entry:
      St_TDrill_11 = false;
      during:
      % N16: peca retirada pela garra da HD2, reseta o ciclo
      if Sensors_90.O_90_Claw_Del && Sensors_90.O_90_Claw_Low && Sensors_90.O_90_Part_in_Claw
      St_TDrill_11 = true;
      else
      St_TDrill_11 = false;
      end
    state Config_TDrill
      entry:
      St_TDrill_1 = false;
      during:
      % FB5 Test + Drill - bloco ativo so neste modo
      if Control_100.C_105_TestDrill && ~Control_100.C_105_Test && ~Control_100.C_105_Rotation
      St_TDrill_1 = true;
      else
      St_TDrill_1 = false;
      end
    state Aguarda_TDrill
      entry:
      St_TDrill_2 = false;
      during:
      % N1: condicoes para iniciar teste+furacao
      if Sensors_100.O_100_PInit_Pos && Sensors_90.O_90_Claw_High && Sensors_100.O_100_RT_Sensor && ~Actuators_100.F_102_RT_On
      St_TDrill_2 = true;
      else
      St_TDrill_2 = false;
      end
    state GiraTeste_TDrill
      entry:
      St_TDrill_3 = false;
      during:
      % N2: mesa girando ate posicao de teste (C6, preset 4)
      if Actuators_100.F_102_RT_On
      St_TDrill_3 = true;
      else
      St_TDrill_3 = false;
      end
    state PosTeste_TDrill
      entry:
      St_TDrill_4 = false;
      during:
      % N3: peca na posicao de teste, temporizador de 2s
      if ~Actuators_100.F_102_RT_On && Sensors_100.O_100_PTest_Pos && Sensors_100.O_100_RT_Sensor
      St_TDrill_4 = true;
      else
      St_TDrill_4 = false;
      end
    state Testando_TDrill
      entry:
      St_TDrill_5 = false;
      during:
      % N4: pino de teste acionado
      if Actuators_100.F_102_Test_Pin
      St_TDrill_5 = true;
      else
      St_TDrill_5 = false;
      end
    state Resultado_TDrill
      entry:
      St_TDrill_6 = false;
      during:
      % N5/N6: resultado do teste no Profibus
      if Control_100.C_105_Test_Ok || Control_100.C_105_Test_Fail
      St_TDrill_6 = true;
      else
      St_TDrill_6 = false;
      end
    state GiraFuro_TDrill
      entry:
      St_TDrill_7 = false;
      during:
      % N7: so gira ate a furadeira se o teste passou (C7, preset 1)
      if Control_100.C_105_Test_Ok && Actuators_100.F_102_RT_On
      St_TDrill_7 = true;
      else
      St_TDrill_7 = false;
      end
    state DesceFuro_TDrill
      entry:
      St_TDrill_8 = false;
      during:
      % N8/N9: trava a peca e desce a furadeira ate o fim de curso
      if Actuators_100.F_102_Drill_Pin && Actuators_100.F_102_Drill_Down && Sensors_100.O_100_SDrill_Low
      St_TDrill_8 = true;
      else
      St_TDrill_8 = false;
      end
    state Furando_TDrill
      entry:
      St_TDrill_9 = false;
      during:
      % N10/N11/N12: fura, sobe e libera o pino
      if Actuators_100.F_102_Drill_On || (Actuators_100.F_102_Drill_Up && Sensors_100.O_100_SDrill_High)
      St_TDrill_9 = true;
      else
      St_TDrill_9 = false;
      end
    state GiraEntrega_TDrill
      entry:
      St_TDrill_10 = false;
      during:
      % N13/N14/N15: gira ate a entrega (C8 se OK, C9 se falha) e libera a peca
      if ~Actuators_100.F_102_RT_On && Sensors_100.O_100_PInit_Pos
      St_TDrill_10 = true;
      else
      St_TDrill_10 = false;
      end
    (default) -> Config_TDrill
    Config_TDrill -> Aguarda_TDrill : [St_TDrill_1 == true]
    Testando_TDrill -> Resultado_TDrill : [St_TDrill_5 == true]
    GiraFuro_TDrill -> DesceFuro_TDrill : [St_TDrill_7 == true]
    DesceFuro_TDrill -> Furando_TDrill : [St_TDrill_8 == true]
    Aguarda_TDrill -> GiraTeste_TDrill : [St_TDrill_2 == true]
    Resultado_TDrill -> GiraFuro_TDrill : [St_TDrill_6 == true]
    PosTeste_TDrill -> Testando_TDrill : [St_TDrill_4 == true && (Actuators_100.F_102_Test_Pin == true || after(2, sec))]
    Furando_TDrill -> GiraEntrega_TDrill : [St_TDrill_9 == true]
    GiraTeste_TDrill -> PosTeste_TDrill : [St_TDrill_3 == true]
    GiraEntrega_TDrill -> Retirada_TDrill : [St_TDrill_10 == true]
  state SRB
    entry:
    StatusSRB_5 = false;   % v0.4.29: zera o fim de ciclo anterior
    state STATE1
      entry:
      StatusSRB_1 = false;
      during:
      % Configuracao da estacao: so este bloco fica ativo se o bit dele estiver ligado
      if Control_60.C_65_SRB_Output
      StatusSRB_1 = true;
      else
      StatusSRB_1 = false;
      end
    state ESTATE2
      entry:
      StatusSRB_2 = false;
      during:
      % Janela de identificacao da peca (T1 = 2s no ladder)
      if Control_50.C_55_PD_Sort
      StatusSRB_2 = true;
      else
      StatusSRB_2 = false;
      end
    state ESTATE3
      entry:
      StatusSRB_3 = false;
      during:
      % Prata: SL1 avanca | Vermelha: SL2 avanca | Preta: ambas recuadas
      if ((~Control_60.C_65_ID_1 && Control_60.C_65_ID_2) && Sensors_60.O_60_SL1_Fwd) || ...
      ((Control_60.C_65_ID_1 && Control_60.C_65_ID_2) && Sensors_60.O_60_SL2_Fwd) || ...
      ((Control_60.C_65_ID_1 && ~Control_60.C_65_ID_2) && Sensors_60.O_60_SL1_Bck && Sensors_60.O_60_SL2_Bck)
      StatusSRB_3 = true;
      else
      StatusSRB_3 = false;
      end
    state ESTATE4
      entry:
      % captura no mesmo passo da entrada
      StatusSRB_4 = Actuators_60.F_62_Identify;
      during:
      % Pino de identificacao acionado (LEITURA do CLP - sombra nao comanda)
      % latch (v0.4.31): o pino desliga junto com o Part_Pass, uma vez observado nao volta a false
      if Actuators_60.F_62_Identify
      StatusSRB_4 = true;
      end
    state ESTATE5
      entry:
      StatusSRB_5 = false;
      during:
      % Pino recuado: ciclo concluido, pronto para a proxima peca
      if ~Actuators_60.F_62_Identify
      StatusSRB_5 = true;
      else
      StatusSRB_5 = false;
      end
    (default) -> SRB.STATE1
    SRB.ESTATE3 -> SRB.ESTATE4 : [StatusSRB_3 == true]
    SRB.ESTATE4 -> SRB.ESTATE5 : [(Sensors_60.O_60_Part_Pass == true || Actuators_60.F_62_Identify == false) && StatusSRB_4 == true]
    SRB.ESTATE2 -> SRB.ESTATE3 : [(Control_60.C_65_ID_1 == true || Control_60.C_65_ID_2 == true || after(2, sec)) && StatusSRB_2 == true]
    SRB.STATE1 -> SRB.ESTATE2 : [Control_50.C_55_PD_Sort == true && StatusSRB_1 == true]
  state Retrieve
    state Config_Retr
      entry:
      St_Retr_1 = false;
      during:
      % FB5 Retrieve Part - bloco ativo so no modo recuperar
      if Control_40.C_45_Initialization && Control_40.C_45_RetrievePart
      St_Retr_1 = true;
      else
      St_Retr_1 = false;
      end
    state Aguarda_Retr
      entry:
      St_Retr_2 = false;
      during:
      % OB1 N5: carro chegou e comando de recuperar presente
      if (Control_40.C_45_Start || (AS_i_40.A_44_CRoute_In && Sensors_40.O_41_Key_Pos)) && AS_i_40.A_44_Cart_Stat
      St_Retr_2 = true;
      else
      St_Retr_2 = false;
      end
    state Recuperando_Retr
      entry:
      St_Retr_3 = false;
      during:
      % FB5 N1: temporizador simulado T2 = 5s (S5T#5S)
      % A estacao nao tem mecanica real: o CLP so conta o tempo.
      if Control_40.C_45_RetrievePart
      St_Retr_3 = true;
      else
      St_Retr_3 = false;
      end
    state ProcessoOK_Retr
      entry:
      St_Retr_4 = false;
      during:
      % OB1 N6: fim do procedimento, sinaliza processo concluido
      if Control_40.C_45_RetrievePart
      St_Retr_4 = true;
      else
      St_Retr_4 = false;
      end
    state LiberaCarro_Retr
      entry:
      St_Retr_5 = false;
      during:
      % OB1 N7: pulso de 2s libera o carro (A_44_CRoute_Out)
      if AS_i_40.A_44_CRoute_Out || ~AS_i_40.A_44_Cart_Stat
      St_Retr_5 = true;
      else
      St_Retr_5 = false;
      end
    (default) -> Config_Retr
    Config_Retr -> Aguarda_Retr : [St_Retr_1 == true]
    Aguarda_Retr -> Recuperando_Retr : [St_Retr_2 == true]
    Recuperando_Retr -> ProcessoOK_Retr : [St_Retr_3 == true && after(5, sec)]
    ProcessoOK_Retr -> LiberaCarro_Retr : [St_Retr_4 == true]
  state ProcessingToPart
    entry:
    P2P1_Armed = false;
    St_P2P1_5_10 = false;   % v0.4.30: zera a flag de peca entregue do ciclo anterior
    during:
    % FB5 N1: Part_ready reseta M2.7 -> C_95_PD_Cart vai a 0 no inicio do ciclo.
    % Ver PD_Cart = 0 arma a saida; PD_Cart = 1 depois disso = FB5 concluido (OB1 N8)
    if ~Control_90.C_95_PD_Cart
    P2P1_Armed = true;
    end
    state Config_P2P1
      % Hd2 OB1 N6 (EN do FB5 Del_2_Cart): Init && Profibus && ( (OK_Move && C_95_Del2Cart) || (C_105_Part_ready && ~A_94_Optic) || M2.0 FB5_P2D_Proc )
      % M0.0 -> C_95_Initialization; M0.6 omitido (interno). M2.0 = auto-retencao -> modelada como latch abaixo
      entry:
      % avaliado no MESMO passo da transicao de entrada (guarda C_105_Part_ready == true)
      St_P2P1_5_1 = Control_90.C_95_Initialization && Control_90.C_92_Profibus && ...
      ( Control_90.C_95_Del2Cart || (Control_100.C_105_Part_ready && ~AS_i_90.A_94_Optic) );
      during:
      % latch (M2.0): uma vez habilitado, nao volta a false mesmo que Part_ready caia
      if Control_90.C_95_Initialization && Control_90.C_92_Profibus && ...
      ( Control_90.C_95_Del2Cart || (Control_100.C_105_Part_ready && ~AS_i_90.A_94_Optic) )
      St_P2P1_5_1 = true;
      end
    state GarraNaEntrega_P2P1
      entry:
      % captura no mesmo passo da entrada
      St_P2P1_5_2 = Actuators_90.F_92_Claw_2_Del || Sensors_90.O_90_Claw_Del;
      during:
      % FB5 N2: garante a garra na posicao de entrega
      % latch, como as bobinas S do FB: uma vez observado, nao volta a false
      if Actuators_90.F_92_Claw_2_Del || Sensors_90.O_90_Claw_Del
      St_P2P1_5_2 = true;
      end
    state DescePega_P2P1
      entry:
      % captura no mesmo passo da entrada
      St_P2P1_5_3 = ( Sensors_90.O_90_Claw_Del && Actuators_90.F_92_Claw_Down && Sensors_90.O_90_Claw_Low ) || ...
      ( Sensors_90.O_90_Claw_Del && Sensors_90.O_90_Part_in_Claw );
      during:
      % FB5 N3: desce a garra na entrega (ou: ja esta com a peca na entrega -> a descida ocorreu)
      % latch, como as bobinas S do FB: uma vez observado, nao volta a false
      if ( Sensors_90.O_90_Claw_Del && Actuators_90.F_92_Claw_Down && Sensors_90.O_90_Claw_Low ) || ...
      ( Sensors_90.O_90_Claw_Del && Sensors_90.O_90_Part_in_Claw )
      St_P2P1_5_3 = true;
      end
    state FechaGarra_P2P1
      entry:
      % captura no mesmo passo da entrada
      St_P2P1_5_4 = Actuators_90.F_92_Close_Claw && Sensors_90.O_90_Part_in_Claw;
      during:
      % FB5 N3: fecha a garra e pega a peca
      % latch, como as bobinas S do FB: uma vez observado, nao volta a false
      if Actuators_90.F_92_Close_Claw && Sensors_90.O_90_Part_in_Claw
      St_P2P1_5_4 = true;
      end
    state SobeComPeca_P2P1
      entry:
      % captura no mesmo passo da entrada
      St_P2P1_5_5 = Sensors_90.O_90_Part_in_Claw && Sensors_90.O_90_Claw_High && ~Actuators_90.F_92_Claw_Down;
      during:
      % FB5 N4: sobe com a peca
      % latch, como as bobinas S do FB: uma vez observado, nao volta a false
      if Sensors_90.O_90_Part_in_Claw && Sensors_90.O_90_Claw_High && ~Actuators_90.F_92_Claw_Down
      St_P2P1_5_5 = true;
      end
    state MoveParaCarro_P2P1
      entry:
      % captura no mesmo passo da entrada
      St_P2P1_5_6 = Sensors_90.O_90_Claw_Cart && Sensors_90.O_90_Part_in_Claw;
      during:
      % FB5 N4: braco chegou ao carro com a peca (F_92_Claw_2_Cart cai ao chegar, por isso nao entra)
      % latch, como as bobinas S do FB: uma vez observado, nao volta a false
      if Sensors_90.O_90_Claw_Cart && Sensors_90.O_90_Part_in_Claw
      St_P2P1_5_6 = true;
      end
    state DesceEntrega_P2P1
      entry:
      % captura no mesmo passo da entrada
      St_P2P1_5_7 = ( Sensors_90.O_90_Claw_Cart && Actuators_90.F_92_Claw_Down && Sensors_90.O_90_Claw_Low ) || ...
      ( Sensors_90.O_90_Claw_Cart && ~Sensors_90.O_90_Part_in_Claw );
      during:
      % FB5 N5: desce sobre o carro (ou: ja soltou a peca no carro -> a descida ocorreu)
      % latch, como as bobinas S do FB: uma vez observado, nao volta a false
      if ( Sensors_90.O_90_Claw_Cart && Actuators_90.F_92_Claw_Down && Sensors_90.O_90_Claw_Low ) || ...
      ( Sensors_90.O_90_Claw_Cart && ~Sensors_90.O_90_Part_in_Claw )
      St_P2P1_5_7 = true;
      end
    state AbreGarra_P2P1
      entry:
      % captura no mesmo passo da entrada
      St_P2P1_5_8 = ~Actuators_90.F_92_Close_Claw && ~Sensors_90.O_90_Part_in_Claw;
      during:
      % FB5 N5: abre a garra e solta a peca no carro
      % latch, como as bobinas S do FB: uma vez observado, nao volta a false
      if ~Actuators_90.F_92_Close_Claw && ~Sensors_90.O_90_Part_in_Claw
      St_P2P1_5_8 = true;
      end
    state SobeVazia_P2P1
      entry:
      % captura no mesmo passo da entrada
      St_P2P1_5_9 = Sensors_90.O_90_Claw_High && ~Sensors_90.O_90_Part_in_Claw;
      during:
      % FB5 N6: sobe sem a peca
      % latch, como as bobinas S do FB: uma vez observado, nao volta a false
      if Sensors_90.O_90_Claw_High && ~Sensors_90.O_90_Part_in_Claw
      St_P2P1_5_9 = true;
      end
    state PecaEntregue_P2P1
      entry:
      % captura no mesmo passo da entrada
      St_P2P1_5_10 = Control_90.C_95_PD_Cart;
      during:
      % FB5 N6: sinaliza peca entregue no carro
      % latch, como as bobinas S do FB: uma vez observado, nao volta a false
      if Control_90.C_95_PD_Cart
      St_P2P1_5_10 = true;
      end
    (default) -> Config_P2P1
    Config_P2P1 -> GarraNaEntrega_P2P1 : [St_P2P1_5_1 == true]
    GarraNaEntrega_P2P1 -> DescePega_P2P1 : [St_P2P1_5_2 == true]
    DescePega_P2P1 -> FechaGarra_P2P1 : [St_P2P1_5_3 == true]
    FechaGarra_P2P1 -> SobeComPeca_P2P1 : [St_P2P1_5_4 == true]
    SobeComPeca_P2P1 -> MoveParaCarro_P2P1 : [St_P2P1_5_5 == true]
    MoveParaCarro_P2P1 -> DesceEntrega_P2P1 : [St_P2P1_5_6 == true]
    DesceEntrega_P2P1 -> AbreGarra_P2P1 : [St_P2P1_5_7 == true]
    AbreGarra_P2P1 -> SobeVazia_P2P1 : [St_P2P1_5_8 == true]
    SobeVazia_P2P1 -> PecaEntregue_P2P1 : [St_P2P1_5_9 == true]
  state Processing_RotationOnly
    state Config_ROnly
      entry:
      St_ROnly_1 = false;
      during:
      % FB6 Rotation Only - bloco ativo so neste modo
      if Control_100.C_105_Rotation && ~Control_100.C_105_Test && ~Control_100.C_105_TestDrill
      St_ROnly_1 = true;
      else
      St_ROnly_1 = false;
      end
    state Aguarda_ROnly
      entry:
      St_ROnly_2 = false;
      during:
      % N1: condicoes para iniciar a rotacao
      if Sensors_100.O_100_PInit_Pos && Sensors_90.O_90_Claw_High && ~Actuators_100.F_102_RT_On
      St_ROnly_2 = true;
      else
      St_ROnly_2 = false;
      end
    state Girando_ROnly
      entry:
      St_ROnly_3 = false;
      during:
      % N2: mesa girando (contador C10, preset 6)
      if Actuators_100.F_102_RT_On
      St_ROnly_3 = true;
      else
      St_ROnly_3 = false;
      end
    state RotacaoOK_ROnly
      entry:
      St_ROnly_4 = false;
      during:
      % N3/N4: fim da rotacao, peca pronta para retirada
      if ~Actuators_100.F_102_RT_On && Sensors_100.O_100_PInit_Pos
      St_ROnly_4 = true;
      else
      St_ROnly_4 = false;
      end
    state Retirada_ROnly
      entry:
      St_ROnly_5 = false;
      during:
      % N5: peca retirada pela garra da HD2, reseta o ciclo
      if Sensors_90.O_90_Claw_Del && Sensors_90.O_90_Claw_Low && Sensors_90.O_90_Part_in_Claw
      St_ROnly_5 = true;
      else
      St_ROnly_5 = false;
      end
    (default) -> Config_ROnly
    Config_ROnly -> Aguarda_ROnly : [St_ROnly_1 == true]
    Aguarda_ROnly -> Girando_ROnly : [St_ROnly_2 == true]
    RotacaoOK_ROnly -> Retirada_ROnly : [St_ROnly_4 == true]
    Girando_ROnly -> RotacaoOK_ROnly : [St_ROnly_3 == true]
  note: Conveyor
  note: Conveyor
  state SBR
    entry:
    StatusSBR_5 = false;   % v0.4.29: zera o fim de ciclo anterior
    state ESTATE3
      entry:
      StatusSBR_3 = false;
      during:
      % Prata: SL1 avanca | Preta: SL2 avanca | Vermelha: ambas recuadas
      if ((~Control_60.C_65_ID_1 && Control_60.C_65_ID_2) && Sensors_60.O_60_SL1_Fwd) || ...
      ((Control_60.C_65_ID_1 && ~Control_60.C_65_ID_2) && Sensors_60.O_60_SL2_Fwd) || ...
      ((Control_60.C_65_ID_1 && Control_60.C_65_ID_2) && Sensors_60.O_60_SL1_Bck && Sensors_60.O_60_SL2_Bck)
      StatusSBR_3 = true;
      else
      StatusSBR_3 = false;
      end
    state STATE1
      entry:
      StatusSBR_1 = false;
      during:
      % Configuracao da estacao: so este bloco fica ativo se o bit dele estiver ligado
      if Control_60.C_65_SBR_Output
      StatusSBR_1 = true;
      else
      StatusSBR_1 = false;
      end
    state ESTATE2
      entry:
      StatusSBR_2 = false;
      during:
      % Janela de identificacao da peca (T1 = 2s no ladder)
      if Control_50.C_55_PD_Sort
      StatusSBR_2 = true;
      else
      StatusSBR_2 = false;
      end
    state ESTATE4
      entry:
      % captura no mesmo passo da entrada
      StatusSBR_4 = Actuators_60.F_62_Identify;
      during:
      % Pino de identificacao acionado (LEITURA do CLP - sombra nao comanda)
      % latch (v0.4.31): o pino desliga junto com o Part_Pass, uma vez observado nao volta a false
      if Actuators_60.F_62_Identify
      StatusSBR_4 = true;
      end
    state ESTATE5
      entry:
      StatusSBR_5 = false;
      during:
      % Pino recuado: ciclo concluido, pronto para a proxima peca
      if ~Actuators_60.F_62_Identify
      StatusSBR_5 = true;
      else
      StatusSBR_5 = false;
      end
    (default) -> SBR.STATE1
    SBR.ESTATE4 -> SBR.ESTATE5 : [(Sensors_60.O_60_Part_Pass == true || Actuators_60.F_62_Identify == false) && StatusSBR_4 == true]
    SBR.ESTATE3 -> SBR.ESTATE4 : [StatusSBR_3 == true]
    SBR.ESTATE2 -> SBR.ESTATE3 : [(Control_60.C_65_ID_1 == true || Control_60.C_65_ID_2 == true || after(2, sec)) && StatusSBR_2 == true]
    SBR.STATE1 -> SBR.ESTATE2 : [Control_50.C_55_PD_Sort == true && StatusSBR_1 == true]
  note: Vision
  state Vision
    entry:
    St_Visn_3 = false;   % v0.4.27: zera a flag de saida do ciclo anterior
    Vis_Req27 = Control_20.C_27_Request;
    Vis_RIn = Control_20.C_26_CRoute_In;
    Vis_ROut = Control_20.C_26_CRoute_Out;
    % Entrada via C_26_CartDel: FB11 N20/N21 so gera CartDel com I14.4 Visi_Cart_Stat -> carro esta na Vision
    Vis_Cart = true;
    during:
    % Master FB11 N22: C_27_Request SETA M4.0 (bobina S) -> o CLP guarda o pedido mesmo que o sinal caia.
    if Control_20.C_27_Request
    Vis_Req27 = true;
    end
    % Master FB2 N31: Q26.2 C_26_CRoute_In (OPC Route Arrive) -> Q23.6 A_23_CRoute_In (Route Arrive Vision)
    if Control_20.C_26_CRoute_In
    Vis_RIn = true;
    end
    % Master FB2 N32: I23.6 A_23_CRoute_Out (Route Depart Vision) OU T9 S_ODT 1s com A_23_CRoute_In -> I26.7 C_26_CRoute_Out
    if Control_20.C_26_CRoute_Out
    Vis_ROut = true;
    end
    state Config_Visn
      entry:
      % captura no mesmo passo da entrada
      St_Visn_1 = Control_20.C_26_CartDel || Sensors_20.O_26_Cart_Stat || Vis_RIn || Vis_ROut;
      during:
      % Carro na Vision: FB11 N20/N21 (C_26_CartDel, pulso 3 s T3) ou FB2 N25 (O_26_Cart_Stat)
      % ou o roteamento da Vision ja comecou (FB2 N31/N32)
      % latch: uma vez observado, nao volta a false
      if Control_20.C_26_CartDel || Sensors_20.O_26_Cart_Stat || Vis_RIn || Vis_ROut
      St_Visn_1 = true;
      end
    state Inspecao_Visn
      entry:
      % captura no mesmo passo da entrada
      St_Visn_2 = Control_20.C_26_CRoute_Out || Vis_ROut;
      during:
      % Inspecao: OPC envia C_26_CRoute_In (Q26.2) -> A_23_CRoute_In (Route Arrive Vision), FB2 N31.
      % Fim da inspecao: A_23_CRoute_Out (Route Depart, I23.6) ou T9 (S_ODT 1 s) -> C_26_CRoute_Out (I26.7), FB2 N32.
      % (substitui a passagem simbolica de 5 s da v4.25)
      % latch: uma vez observado, nao volta a false
      if Control_20.C_26_CRoute_Out || Vis_ROut
      St_Visn_2 = true;
      end
    state FinishesProcess_Visn
      entry:
      % captura no mesmo passo da entrada
      St_Visn_3 = Control_20.C_27_Request || Vis_Req27;
      during:
      %% Inspecao concluida: aguarda o pedido de carrinho do Robot (C_27_Request, visto agora ou antes)
      % latch: uma vez observado, nao volta a false
      if Control_20.C_27_Request || Vis_Req27
      St_Visn_3 = true;
      end
    (default) -> Config_Visn
    Inspecao_Visn -> FinishesProcess_Visn : [St_Visn_2 == true || Vis_Req27 == true]
    Config_Visn -> Inspecao_Visn : [St_Visn_1 == true]
  note: Robot [30]
  state Robot1
    state Config_Rbt1
      entry:
      St_Rbt1_1 = false;
      during:
      % FB3 Robot Remote (Master) - modo 1
      % N15: os modos sao mutuamente exclusivos
      if Control_30.C_30_Robot1
      St_Rbt1_1 = false;
      else
      St_Rbt1_1 = false;
      end
      if Control_30.C_30_Robot1
      St_Rbt1_1 = true;
      end
    state AguardaCarro_Rbt1
      entry:
      St_Rbt1_2 = false;
      during:
      % N10/N11: carro na estacao, com peca, sensor optico
      if AS_i_30.A_34_Cart_Stat && ~AS_i_30.A_34_No_Cart && AS_i_30.A_34_Optic
      St_Rbt1_2 = true;
      else
      St_Rbt1_2 = false;
      end
    state PegaPeca_Rbt1
      entry:
      St_Rbt1_3 = false;
      during:
      % N8: cilindro da mola avanca para pegar a peca
      if Actuators_30.F_33_Spring_Cyl && Sensors_30.O_32_Sp_Cyl_Fwd && Sensors_30.O_31_Part_in_Claw
      St_Rbt1_3 = true;
      else
      St_Rbt1_3 = false;
      end
    state ColocaTampa_Rbt1
      entry:
      St_Rbt1_4 = false;
      during:
      % N9: cilindro da tampa avanca (magazine nao pode estar vazio)
      if Actuators_30.F_33_Cover_Cyl && Sensors_30.O_32_Co_Cyl_Fwd && ~Sensors_30.O_32_CoMag_Empty
      St_Rbt1_4 = true;
      else
      St_Rbt1_4 = false;
      end
    state Recua_Rbt1
      entry:
      St_Rbt1_5 = false;
      during:
      % N8/N9: os dois cilindros recuam para a posicao de pick-up
      if Sensors_30.O_32_Sp_Cyl_Bck && Sensors_30.O_32_Co_Cyl_Bck && Sensors_30.O_32_Sp_PickUp && Sensors_30.O_32_Co_PickUp
      St_Rbt1_5 = true;
      else
      St_Rbt1_5 = false;
      end
    state PecaEntregue_Rbt1
      entry:
      St_Rbt1_6 = false;
      during:
      % N13: borda de FB3_CartDel sinaliza peca entregue
      if Control_30.C_35_Part_Del
      St_Rbt1_6 = true;
      else
      St_Rbt1_6 = false;
      end
    state LiberaCarro_Rbt1
      entry:
      St_Rbt1_7 = false;
      during:
      % N14: T8 (2s) e processo terminado -> libera o carro
      if AS_i_30.A_34_CRoute_Out || ~AS_i_30.A_34_Cart_Stat
      St_Rbt1_7 = true;
      else
      St_Rbt1_7 = false;
      end
    (default) -> Config_Rbt1
    Config_Rbt1 -> AguardaCarro_Rbt1 : [St_Rbt1_1 == true]
    AguardaCarro_Rbt1 -> PegaPeca_Rbt1 : [St_Rbt1_2 == true]
    PegaPeca_Rbt1 -> ColocaTampa_Rbt1 : [St_Rbt1_3 == true]
    ColocaTampa_Rbt1 -> Recua_Rbt1 : [St_Rbt1_4 == true]
    Recua_Rbt1 -> PecaEntregue_Rbt1 : [St_Rbt1_5 == true && (Control_30.C_35_Part_Del == true || after(5, sec))]
    PecaEntregue_Rbt1 -> LiberaCarro_Rbt1 : [St_Rbt1_6 == true && (AS_i_30.A_34_CRoute_Out == true || after(2, sec))]
  note: Conveyor
  state Robot2
    state Config_Rbt2
      entry:
      St_Rbt2_1 = false;
      during:
      % FB3 Robot Remote (Master) - modo 2
      % N15: os modos sao mutuamente exclusivos
      if Control_30.C_30_Robot2
      St_Rbt2_1 = false;
      else
      St_Rbt2_1 = false;
      end
      if Control_30.C_30_Robot2
      St_Rbt2_1 = true;
      end
    state AguardaCarro_Rbt2
      entry:
      St_Rbt2_2 = false;
      during:
      % N10/N11: carro na estacao, com peca, sensor optico
      if AS_i_30.A_34_Cart_Stat && ~AS_i_30.A_34_No_Cart && AS_i_30.A_34_Optic
      St_Rbt2_2 = true;
      else
      St_Rbt2_2 = false;
      end
    state PegaPeca_Rbt2
      entry:
      St_Rbt2_3 = false;
      during:
      % N8: cilindro da mola avanca para pegar a peca
      if Actuators_30.F_33_Spring_Cyl && Sensors_30.O_32_Sp_Cyl_Fwd && Sensors_30.O_31_Part_in_Claw
      St_Rbt2_3 = true;
      else
      St_Rbt2_3 = false;
      end
    state ColocaTampa_Rbt2
      entry:
      St_Rbt2_4 = false;
      during:
      % N9: cilindro da tampa avanca (magazine nao pode estar vazio)
      if Actuators_30.F_33_Cover_Cyl && Sensors_30.O_32_Co_Cyl_Fwd && ~Sensors_30.O_32_CoMag_Empty
      St_Rbt2_4 = true;
      else
      St_Rbt2_4 = false;
      end
    state Recua_Rbt2
      entry:
      St_Rbt2_5 = false;
      during:
      % N8/N9: os dois cilindros recuam para a posicao de pick-up
      if Sensors_30.O_32_Sp_Cyl_Bck && Sensors_30.O_32_Co_Cyl_Bck && Sensors_30.O_32_Sp_PickUp && Sensors_30.O_32_Co_PickUp
      St_Rbt2_5 = true;
      else
      St_Rbt2_5 = false;
      end
    state PecaEntregue_Rbt2
      entry:
      St_Rbt2_6 = false;
      during:
      % N13: borda de FB3_CartDel sinaliza peca entregue
      if Control_30.C_35_Part_Del
      St_Rbt2_6 = true;
      else
      St_Rbt2_6 = false;
      end
    state LiberaCarro_Rbt2
      entry:
      St_Rbt2_7 = false;
      during:
      % N14: T8 (2s) e processo terminado -> libera o carro
      if AS_i_30.A_34_CRoute_Out || ~AS_i_30.A_34_Cart_Stat
      St_Rbt2_7 = true;
      else
      St_Rbt2_7 = false;
      end
    (default) -> Config_Rbt2
    Config_Rbt2 -> AguardaCarro_Rbt2 : [St_Rbt2_1 == true]
    AguardaCarro_Rbt2 -> PegaPeca_Rbt2 : [St_Rbt2_2 == true]
    PegaPeca_Rbt2 -> ColocaTampa_Rbt2 : [St_Rbt2_3 == true]
    ColocaTampa_Rbt2 -> Recua_Rbt2 : [St_Rbt2_4 == true]
    Recua_Rbt2 -> PecaEntregue_Rbt2 : [St_Rbt2_5 == true && (Control_30.C_35_Part_Del == true || after(5, sec))]
    PecaEntregue_Rbt2 -> LiberaCarro_Rbt2 : [St_Rbt2_6 == true && (AS_i_30.A_34_CRoute_Out == true || after(2, sec))]
  state CartToTesting
    state DeSorting_Cv24
      entry:
      St_Cv24_2a = false;
      during:
      % FB11 N2: abre caminho vindo de Sorting (29) - prioridade 1
      % ordem do ladder: carro mais proximo a montante do laco
      if Control_20.C_24_Request && Sensors_20.O_29_Cart_Stat
      St_Cv24_2a = true;
      else
      St_Cv24_2a = false;
      end
    state DeStorage_Cv24
      entry:
      St_Cv24_2b = false;
      during:
      % FB11 N2: abre caminho vindo de Storage (28) - prioridade 2
      % ordem do ladder: carro mais proximo a montante do laco
      if Control_20.C_24_Request && Sensors_20.O_28_Cart_Stat && ~Sensors_20.O_29_Cart_Stat
      St_Cv24_2b = true;
      else
      St_Cv24_2b = false;
      end
    state Config_Cv24
      entry:
      St_Cv24_1 = false;
      during:
      % FB11 N1: solicitacao de carrinho para Testing
      if Control_20.C_24_Request
      St_Cv24_1 = true;
      else
      St_Cv24_1 = false;
      end
    state EsteiraLigada_Cv24
      entry:
      St_Cv24_3 = false;
      during:
      % FB11 N3: aciona a esteira (exige a controladora ligada)
      if Actuators_20.F_22_Conveyor && Sensors_20.O_20_Controler_On
      St_Cv24_3 = true;
      else
      St_Cv24_3 = false;
      end
    state CarroProximo_Cv24
      entry:
      St_Cv24_4 = false;
      during:
      % FB11 N4: carro proximo da estacao, desliga os pinos
      if Sensors_20.O_24_Cart_Next
      St_Cv24_4 = true;
      else
      St_Cv24_4 = false;
      end
    state IdentificaCarro_Cv24
      entry:
      St_Cv24_5 = false;
      during:
      % FB11 N5: contador identifica o numero do carro
      if Sensors_20.O_24_Count || Sensors_20.O_24_Pist_Bck
      St_Cv24_5 = true;
      else
      St_Cv24_5 = false;
      end
    state CarroChegou_Cv24
      entry:
      St_Cv24_6 = false;
      during:
      % FB11 N6: carro na estacao (T = 3s antes de resetar)
      if Sensors_20.O_24_Cart_Stat && Sensors_20.O_24_Optic
      St_Cv24_6 = true;
      else
      St_Cv24_6 = false;
      end
    state SinalizaChegada_Cv24
      entry:
      St_Cv24_7 = false;
      during:
      % FB11 N7: sinaliza chegada do carro
      if Control_20.C_24_CartDel
      St_Cv24_7 = true;
      else
      St_Cv24_7 = false;
      end
    state DeRobot_Cv24
      entry:
      St_Cv24_2c = false;
      during:
      % FB11 N2: abre caminho vindo de Robot (27) - prioridade 3
      % ordem do ladder: carro mais proximo a montante do laco
      if Control_20.C_24_Request && Sensors_20.O_27_Cart_Stat && ~Sensors_20.O_29_Cart_Stat && ~Sensors_20.O_28_Cart_Stat
      St_Cv24_2c = true;
      else
      St_Cv24_2c = false;
      end
    state DeVision_Cv24
      entry:
      St_Cv24_2d = false;
      during:
      % FB11 N2: abre caminho vindo de Vision (26) - prioridade 4
      % ordem do ladder: carro mais proximo a montante do laco
      if Control_20.C_24_Request && Sensors_20.O_26_Cart_Stat && ~Sensors_20.O_29_Cart_Stat && ~Sensors_20.O_28_Cart_Stat && ~Sensors_20.O_27_Cart_Stat
      St_Cv24_2d = true;
      else
      St_Cv24_2d = false;
      end
    state DeProcessing_Cv24
      entry:
      St_Cv24_2e = false;
      during:
      % FB11 N2: abre caminho vindo de Processing (25) - prioridade 5
      % ordem do ladder: carro mais proximo a montante do laco
      if Control_20.C_24_Request && Sensors_20.O_25_Cart_Stat && ~Sensors_20.O_29_Cart_Stat && ~Sensors_20.O_28_Cart_Stat && ~Sensors_20.O_27_Cart_Stat && ~Sensors_20.O_26_Cart_Stat
      St_Cv24_2e = true;
      else
      St_Cv24_2e = false;
      end
    Config_Cv24 -> DeSorting_Cv24 [order 1] : [Control_20.C_24_Request == true && Sensors_20.O_29_Cart_Stat == true]
    DeSorting_Cv24 -> EsteiraLigada_Cv24 : [St_Cv24_2a == true]
    Config_Cv24 -> DeStorage_Cv24 [order 2] : [Control_20.C_24_Request == true && Sensors_20.O_28_Cart_Stat == true && Sensors_20.O_29_Cart_Stat == false]
    (default) -> Config_Cv24
    DeStorage_Cv24 -> EsteiraLigada_Cv24 : [St_Cv24_2b == true]
    DeRobot_Cv24 -> EsteiraLigada_Cv24 : [St_Cv24_2c == true]
    EsteiraLigada_Cv24 -> CarroProximo_Cv24 : [St_Cv24_3 == true]
    CarroProximo_Cv24 -> IdentificaCarro_Cv24 : [St_Cv24_4 == true]
    IdentificaCarro_Cv24 -> CarroChegou_Cv24 : [St_Cv24_5 == true]
    DeProcessing_Cv24 -> EsteiraLigada_Cv24 : [St_Cv24_2e == true]
    DeVision_Cv24 -> EsteiraLigada_Cv24 : [St_Cv24_2d == true]
    CarroChegou_Cv24 -> SinalizaChegada_Cv24 : [St_Cv24_6 == true && (Control_20.C_24_CartDel == true || after(3, sec))]
    Config_Cv24 -> DeRobot_Cv24 [order 3] : [Control_20.C_24_Request == true && Sensors_20.O_27_Cart_Stat == true && Sensors_20.O_29_Cart_Stat == false && Sensors_20.O_28_Cart_Stat == false]
    Config_Cv24 -> DeVision_Cv24 [order 4] : [Control_20.C_24_Request == true && Sensors_20.O_26_Cart_Stat == true && Sensors_20.O_29_Cart_Stat == false && Sensors_20.O_28_Cart_Stat == false && Sensors_20.O_27_Cart_Stat == false]
    Config_Cv24 -> DeProcessing_Cv24 [order 5] : [Control_20.C_24_Request == true && Sensors_20.O_25_Cart_Stat == true && Sensors_20.O_29_Cart_Stat == false && Sensors_20.O_28_Cart_Stat == false && Sensors_20.O_27_Cart_Stat == false && Sensors_20.O_26_Cart_Stat == false]
  state CartToProcessing
    state DeTesting_Cv25
      entry:
      St_Cv25_2a = false;
      during:
      % FB11 N2: abre caminho vindo de Testing (24) - prioridade 1
      % ordem do ladder: carro mais proximo a montante do laco
      if Control_20.C_25_Request && Sensors_20.O_24_Cart_Stat
      St_Cv25_2a = true;
      else
      St_Cv25_2a = false;
      end
    state DeSorting_Cv25
      entry:
      St_Cv25_2b = false;
      during:
      % FB11 N2: abre caminho vindo de Sorting (29) - prioridade 2
      % ordem do ladder: carro mais proximo a montante do laco
      if Control_20.C_25_Request && Sensors_20.O_29_Cart_Stat && ~Sensors_20.O_24_Cart_Stat
      St_Cv25_2b = true;
      else
      St_Cv25_2b = false;
      end
    state Config_Cv25
      entry:
      St_Cv25_1 = false;
      during:
      % FB11 N1: solicitacao de carrinho para Processing
      if Control_20.C_25_Request
      St_Cv25_1 = true;
      else
      St_Cv25_1 = false;
      end
    state EsteiraLigada_Cv25
      entry:
      St_Cv25_3 = false;
      during:
      % FB11 N3: aciona a esteira (exige a controladora ligada)
      if Actuators_20.F_22_Conveyor && Sensors_20.O_20_Controler_On
      St_Cv25_3 = true;
      else
      St_Cv25_3 = false;
      end
    state CarroProximo_Cv25
      entry:
      St_Cv25_4 = false;
      during:
      % FB11 N4: carro proximo da estacao, desliga os pinos
      if Sensors_20.O_25_Cart_Next
      St_Cv25_4 = true;
      else
      St_Cv25_4 = false;
      end
    state IdentificaCarro_Cv25
      entry:
      St_Cv25_5 = false;
      during:
      % FB11 N5: contador identifica o numero do carro
      if Sensors_20.O_25_Count || Sensors_20.O_25_Pist_Bck
      St_Cv25_5 = true;
      else
      St_Cv25_5 = false;
      end
    state CarroChegou_Cv25
      entry:
      St_Cv25_6 = false;
      during:
      % FB11 N6: carro na estacao (T = 3s antes de resetar)
      if Sensors_20.O_25_Cart_Stat && Sensors_20.O_25_Optic
      St_Cv25_6 = true;
      else
      St_Cv25_6 = false;
      end
    state SinalizaChegada_Cv25
      entry:
      St_Cv25_7 = false;
      during:
      % FB11 N7: sinaliza chegada do carro
      if Control_20.C_25_CartDel
      St_Cv25_7 = true;
      else
      St_Cv25_7 = false;
      end
    state DeStorage_Cv25
      entry:
      St_Cv25_2c = false;
      during:
      % FB11 N2: abre caminho vindo de Storage (28) - prioridade 3
      % ordem do ladder: carro mais proximo a montante do laco
      if Control_20.C_25_Request && Sensors_20.O_28_Cart_Stat && ~Sensors_20.O_24_Cart_Stat && ~Sensors_20.O_29_Cart_Stat
      St_Cv25_2c = true;
      else
      St_Cv25_2c = false;
      end
    state DeRobot_Cv25
      entry:
      St_Cv25_2d = false;
      during:
      % FB11 N2: abre caminho vindo de Robot (27) - prioridade 4
      % ordem do ladder: carro mais proximo a montante do laco
      if Control_20.C_25_Request && Sensors_20.O_27_Cart_Stat && ~Sensors_20.O_24_Cart_Stat && ~Sensors_20.O_29_Cart_Stat && ~Sensors_20.O_28_Cart_Stat
      St_Cv25_2d = true;
      else
      St_Cv25_2d = false;
      end
    state DeVision_Cv25
      entry:
      St_Cv25_2e = false;
      during:
      % FB11 N2: abre caminho vindo de Vision (26) - prioridade 5
      % ordem do ladder: carro mais proximo a montante do laco
      if Control_20.C_25_Request && Sensors_20.O_26_Cart_Stat && ~Sensors_20.O_24_Cart_Stat && ~Sensors_20.O_29_Cart_Stat && ~Sensors_20.O_28_Cart_Stat && ~Sensors_20.O_27_Cart_Stat
      St_Cv25_2e = true;
      else
      St_Cv25_2e = false;
      end
    Config_Cv25 -> DeTesting_Cv25 [order 1] : [Control_20.C_25_Request == true && Sensors_20.O_24_Cart_Stat == true]
    DeTesting_Cv25 -> EsteiraLigada_Cv25 : [St_Cv25_2a == true]
    Config_Cv25 -> DeSorting_Cv25 [order 2] : [Control_20.C_25_Request == true && Sensors_20.O_29_Cart_Stat == true && Sensors_20.O_24_Cart_Stat == false]
    DeSorting_Cv25 -> EsteiraLigada_Cv25 : [St_Cv25_2b == true]
    (default) -> Config_Cv25
    DeStorage_Cv25 -> EsteiraLigada_Cv25 : [St_Cv25_2c == true]
    Config_Cv25 -> DeStorage_Cv25 [order 3] : [Control_20.C_25_Request == true && Sensors_20.O_28_Cart_Stat == true && Sensors_20.O_24_Cart_Stat == false && Sensors_20.O_29_Cart_Stat == false]
    DeRobot_Cv25 -> EsteiraLigada_Cv25 : [St_Cv25_2d == true]
    DeVision_Cv25 -> EsteiraLigada_Cv25 : [St_Cv25_2e == true]
    EsteiraLigada_Cv25 -> CarroProximo_Cv25 : [St_Cv25_3 == true]
    CarroProximo_Cv25 -> IdentificaCarro_Cv25 : [St_Cv25_4 == true]
    IdentificaCarro_Cv25 -> CarroChegou_Cv25 : [St_Cv25_5 == true]
    CarroChegou_Cv25 -> SinalizaChegada_Cv25 : [St_Cv25_6 == true && (Control_20.C_25_CartDel == true || after(3, sec))]
    Config_Cv25 -> DeVision_Cv25 [order 5] : [Control_20.C_25_Request == true && Sensors_20.O_26_Cart_Stat == true && Sensors_20.O_24_Cart_Stat == false && Sensors_20.O_29_Cart_Stat == false && Sensors_20.O_28_Cart_Stat == false && Sensors_20.O_27_Cart_Stat == false]
    Config_Cv25 -> DeRobot_Cv25 [order 4] : [Control_20.C_25_Request == true && Sensors_20.O_27_Cart_Stat == true && Sensors_20.O_24_Cart_Stat == false && Sensors_20.O_29_Cart_Stat == false && Sensors_20.O_28_Cart_Stat == false]
  state CartToProcessing1
    state DeProcessing_Cv26
      entry:
      St_Cv26_2a = false;
      during:
      % FB11 N2: abre caminho vindo de Processing (25) - prioridade 1
      % ordem do ladder: carro mais proximo a montante do laco
      if Control_20.C_26_Request && Sensors_20.O_25_Cart_Stat
      St_Cv26_2a = true;
      else
      St_Cv26_2a = false;
      end
    state DeTesting_Cv26
      entry:
      St_Cv26_2b = false;
      during:
      % FB11 N2: abre caminho vindo de Testing (24) - prioridade 2
      % ordem do ladder: carro mais proximo a montante do laco
      if Control_20.C_26_Request && Sensors_20.O_24_Cart_Stat && ~Sensors_20.O_25_Cart_Stat
      St_Cv26_2b = true;
      else
      St_Cv26_2b = false;
      end
    state Config_Cv26
      entry:
      St_Cv26_1 = false;
      during:
      % FB11 N1: solicitacao de carrinho para Vision
      if Control_20.C_26_Request
      St_Cv26_1 = true;
      else
      St_Cv26_1 = false;
      end
    state EsteiraLigada_Cv26
      entry:
      St_Cv26_3 = false;
      during:
      % FB11 N3: aciona a esteira (exige a controladora ligada)
      if Actuators_20.F_22_Conveyor && Sensors_20.O_20_Controler_On
      St_Cv26_3 = true;
      else
      St_Cv26_3 = false;
      end
    state CarroProximo_Cv26
      entry:
      St_Cv26_4 = false;
      during:
      % FB11 N4: carro proximo da estacao, desliga os pinos
      if Sensors_20.O_26_Cart_Next
      St_Cv26_4 = true;
      else
      St_Cv26_4 = false;
      end
    state IdentificaCarro_Cv26
      entry:
      St_Cv26_5 = false;
      during:
      % FB11 N5: contador identifica o numero do carro
      if Sensors_20.O_26_Count || Sensors_20.O_26_Pist_Bck
      St_Cv26_5 = true;
      else
      St_Cv26_5 = false;
      end
    state CarroChegou_Cv26
      entry:
      St_Cv26_6 = false;
      during:
      % FB11 N6: carro na estacao (T = 3s antes de resetar)
      if Sensors_20.O_26_Cart_Stat && Sensors_20.O_26_Optic
      St_Cv26_6 = true;
      else
      St_Cv26_6 = false;
      end
    state SinalizaChegada_Cv26
      entry:
      St_Cv26_7 = false;
      during:
      % FB11 N7: sinaliza chegada do carro
      if Control_20.C_26_CartDel
      St_Cv26_7 = true;
      else
      St_Cv26_7 = false;
      end
    state DeSorting_Cv26
      entry:
      St_Cv26_2c = false;
      during:
      % FB11 N2: abre caminho vindo de Sorting (29) - prioridade 3
      % ordem do ladder: carro mais proximo a montante do laco
      if Control_20.C_26_Request && Sensors_20.O_29_Cart_Stat && ~Sensors_20.O_25_Cart_Stat && ~Sensors_20.O_24_Cart_Stat
      St_Cv26_2c = true;
      else
      St_Cv26_2c = false;
      end
    state DeStorage_Cv26
      entry:
      St_Cv26_2d = false;
      during:
      % FB11 N2: abre caminho vindo de Storage (28) - prioridade 4
      % ordem do ladder: carro mais proximo a montante do laco
      if Control_20.C_26_Request && Sensors_20.O_28_Cart_Stat && ~Sensors_20.O_25_Cart_Stat && ~Sensors_20.O_24_Cart_Stat && ~Sensors_20.O_29_Cart_Stat
      St_Cv26_2d = true;
      else
      St_Cv26_2d = false;
      end
    state DeRobot_Cv26
      entry:
      St_Cv26_2e = false;
      during:
      % FB11 N2: abre caminho vindo de Robot (27) - prioridade 5
      % ordem do ladder: carro mais proximo a montante do laco
      if Control_20.C_26_Request && Sensors_20.O_27_Cart_Stat && ~Sensors_20.O_25_Cart_Stat && ~Sensors_20.O_24_Cart_Stat && ~Sensors_20.O_29_Cart_Stat && ~Sensors_20.O_28_Cart_Stat
      St_Cv26_2e = true;
      else
      St_Cv26_2e = false;
      end
    Config_Cv26 -> DeProcessing_Cv26 [order 1] : [Control_20.C_26_Request == true && Sensors_20.O_25_Cart_Stat == true]
    DeProcessing_Cv26 -> EsteiraLigada_Cv26 : [St_Cv26_2a == true]
    Config_Cv26 -> DeTesting_Cv26 [order 2] : [Control_20.C_26_Request == true && Sensors_20.O_24_Cart_Stat == true && Sensors_20.O_25_Cart_Stat == false]
    DeTesting_Cv26 -> EsteiraLigada_Cv26 : [St_Cv26_2b == true]
    DeSorting_Cv26 -> EsteiraLigada_Cv26 : [St_Cv26_2c == true]
    Config_Cv26 -> DeSorting_Cv26 [order 3] : [Control_20.C_26_Request == true && Sensors_20.O_29_Cart_Stat == true && Sensors_20.O_25_Cart_Stat == false && Sensors_20.O_24_Cart_Stat == false]
    DeStorage_Cv26 -> EsteiraLigada_Cv26 : [St_Cv26_2d == true]
    (default) -> Config_Cv26
    DeRobot_Cv26 -> EsteiraLigada_Cv26 : [St_Cv26_2e == true]
    CarroProximo_Cv26 -> IdentificaCarro_Cv26 : [St_Cv26_4 == true]
    EsteiraLigada_Cv26 -> CarroProximo_Cv26 : [St_Cv26_3 == true]
    IdentificaCarro_Cv26 -> CarroChegou_Cv26 : [St_Cv26_5 == true]
    CarroChegou_Cv26 -> SinalizaChegada_Cv26 : [St_Cv26_6 == true && (Control_20.C_26_CartDel == true || after(3, sec))]
    Config_Cv26 -> DeRobot_Cv26 [order 5] : [Control_20.C_26_Request == true && Sensors_20.O_27_Cart_Stat == true && Sensors_20.O_25_Cart_Stat == false && Sensors_20.O_24_Cart_Stat == false && Sensors_20.O_29_Cart_Stat == false && Sensors_20.O_28_Cart_Stat == false]
    Config_Cv26 -> DeStorage_Cv26 [order 4] : [Control_20.C_26_Request == true && Sensors_20.O_28_Cart_Stat == true && Sensors_20.O_25_Cart_Stat == false && Sensors_20.O_24_Cart_Stat == false && Sensors_20.O_29_Cart_Stat == false]
  state CartToProcessing2
    exit:
    Vis_Cart = false;
    state DeVision_Cv27
      entry:
      % captura no mesmo passo da entrada
      St_Cv27_2a = St_Cv27_1 && (Sensors_20.O_26_Cart_Stat || Vis_Cart);
      during:
      % FB11 N2: abre caminho vindo de Vision (26) - prioridade 1
      % Vis_Cart: o carro chegou na Vision (FB11 N20/N21) e o I14.4 pode ja ter caido com a liberacao
      % latch: uma vez observado, nao volta a false
      if St_Cv27_1 && (Sensors_20.O_26_Cart_Stat || Vis_Cart)
      St_Cv27_2a = true;
      end
    state DeProcessing_Cv27
      entry:
      % captura no mesmo passo da entrada
      St_Cv27_2b = St_Cv27_1 && Sensors_20.O_25_Cart_Stat && ~Sensors_20.O_26_Cart_Stat;
      during:
      % FB11 N2: abre caminho vindo de Processing (25) - prioridade 2
      % ordem do ladder: carro mais proximo a montante do laco
      % latch: uma vez observado, nao volta a false
      if St_Cv27_1 && Sensors_20.O_25_Cart_Stat && ~Sensors_20.O_26_Cart_Stat
      St_Cv27_2b = true;
      end
    state Config_Cv27
      entry:
      % captura no mesmo passo da entrada
      St_Cv27_1 = Control_20.C_27_Request || Vis_Req27;
      during:
      % FB11 N1: solicitacao de carrinho para Robot
      % pedido pode ter sido visto ainda na Vision (Vis_Req27) - FB11 N22 guarda em M4.0
      % latch: uma vez observado, nao volta a false
      if Control_20.C_27_Request || Vis_Req27
      St_Cv27_1 = true;
      end
    state EsteiraLigada_Cv27
      entry:
      % captura no mesmo passo da entrada
      St_Cv27_3 = Actuators_20.F_22_Conveyor && Sensors_20.O_20_Controler_On;
      during:
      % FB11 N3: aciona a esteira (exige a controladora ligada)
      % latch: uma vez observado, nao volta a false
      if Actuators_20.F_22_Conveyor && Sensors_20.O_20_Controler_On
      St_Cv27_3 = true;
      end
    state CarroProximo_Cv27
      entry:
      % captura no mesmo passo da entrada
      St_Cv27_4 = Sensors_20.O_27_Cart_Next;
      during:
      % FB11 N4: carro proximo da estacao, desliga os pinos
      % latch: uma vez observado, nao volta a false
      if Sensors_20.O_27_Cart_Next
      St_Cv27_4 = true;
      end
    state IdentificaCarro_Cv27
      entry:
      % captura no mesmo passo da entrada
      St_Cv27_5 = Sensors_20.O_27_Count || Sensors_20.O_27_Pist_Bck;
      during:
      % FB11 N5: contador identifica o numero do carro
      % latch: uma vez observado, nao volta a false
      if Sensors_20.O_27_Count || Sensors_20.O_27_Pist_Bck
      St_Cv27_5 = true;
      end
    state CarroChegou_Cv27
      entry:
      % captura no mesmo passo da entrada
      St_Cv27_6 = Sensors_20.O_27_Cart_Stat && Sensors_20.O_27_Optic;
      during:
      % FB11 N6: carro na estacao (T = 3s antes de resetar)
      % latch: uma vez observado, nao volta a false
      if Sensors_20.O_27_Cart_Stat && Sensors_20.O_27_Optic
      St_Cv27_6 = true;
      end
    state SinalizaChegada_Cv27
      entry:
      % captura no mesmo passo da entrada
      St_Cv27_7 = Control_20.C_27_CartDel;
      during:
      % FB11 N7: sinaliza chegada do carro
      % latch: uma vez observado, nao volta a false
      if Control_20.C_27_CartDel
      St_Cv27_7 = true;
      end
    state DeTesting_Cv27
      entry:
      % captura no mesmo passo da entrada
      St_Cv27_2c = St_Cv27_1 && Sensors_20.O_24_Cart_Stat && ~Sensors_20.O_26_Cart_Stat && ~Sensors_20.O_25_Cart_Stat;
      during:
      % FB11 N2: abre caminho vindo de Testing (24) - prioridade 3
      % ordem do ladder: carro mais proximo a montante do laco
      % latch: uma vez observado, nao volta a false
      if St_Cv27_1 && Sensors_20.O_24_Cart_Stat && ~Sensors_20.O_26_Cart_Stat && ~Sensors_20.O_25_Cart_Stat
      St_Cv27_2c = true;
      end
    state DeSorting_Cv27
      entry:
      % captura no mesmo passo da entrada
      St_Cv27_2d = St_Cv27_1 && Sensors_20.O_29_Cart_Stat && ~Sensors_20.O_26_Cart_Stat && ~Sensors_20.O_25_Cart_Stat && ~Sensors_20.O_24_Cart_Stat;
      during:
      % FB11 N2: abre caminho vindo de Sorting (29) - prioridade 4
      % ordem do ladder: carro mais proximo a montante do laco
      % latch: uma vez observado, nao volta a false
      if St_Cv27_1 && Sensors_20.O_29_Cart_Stat && ~Sensors_20.O_26_Cart_Stat && ~Sensors_20.O_25_Cart_Stat && ~Sensors_20.O_24_Cart_Stat
      St_Cv27_2d = true;
      end
    state DeStorage_Cv27
      entry:
      % captura no mesmo passo da entrada
      St_Cv27_2e = St_Cv27_1 && Sensors_20.O_28_Cart_Stat && ~Sensors_20.O_26_Cart_Stat && ~Sensors_20.O_25_Cart_Stat && ~Sensors_20.O_24_Cart_Stat && ~Sensors_20.O_29_Cart_Stat;
      during:
      % FB11 N2: abre caminho vindo de Storage (28) - prioridade 5
      % ordem do ladder: carro mais proximo a montante do laco
      % latch: uma vez observado, nao volta a false
      if St_Cv27_1 && Sensors_20.O_28_Cart_Stat && ~Sensors_20.O_26_Cart_Stat && ~Sensors_20.O_25_Cart_Stat && ~Sensors_20.O_24_Cart_Stat && ~Sensors_20.O_29_Cart_Stat
      St_Cv27_2e = true;
      end
    Config_Cv27 -> DeVision_Cv27 [order 1] : [St_Cv27_1 == true && (Sensors_20.O_26_Cart_Stat == true || Vis_Cart == true)]
    DeVision_Cv27 -> EsteiraLigada_Cv27 : [St_Cv27_2a == true]
    Config_Cv27 -> DeProcessing_Cv27 [order 2] : [St_Cv27_1 == true && Sensors_20.O_25_Cart_Stat == true && Sensors_20.O_26_Cart_Stat == false]
    DeProcessing_Cv27 -> EsteiraLigada_Cv27 : [St_Cv27_2b == true]
    DeTesting_Cv27 -> EsteiraLigada_Cv27 : [St_Cv27_2c == true]
    (default) -> Config_Cv27
    Config_Cv27 -> DeTesting_Cv27 [order 3] : [St_Cv27_1 == true && Sensors_20.O_24_Cart_Stat == true && Sensors_20.O_26_Cart_Stat == false && Sensors_20.O_25_Cart_Stat == false]
    DeSorting_Cv27 -> EsteiraLigada_Cv27 : [St_Cv27_2d == true]
    DeStorage_Cv27 -> EsteiraLigada_Cv27 : [St_Cv27_2e == true]
    EsteiraLigada_Cv27 -> CarroProximo_Cv27 : [St_Cv27_3 == true]
    IdentificaCarro_Cv27 -> CarroChegou_Cv27 : [St_Cv27_5 == true]
    CarroProximo_Cv27 -> IdentificaCarro_Cv27 : [St_Cv27_4 == true]
    CarroChegou_Cv27 -> SinalizaChegada_Cv27 : [St_Cv27_6 == true && (Control_20.C_27_CartDel == true || after(3, sec))]
    Config_Cv27 -> DeStorage_Cv27 [order 5] : [St_Cv27_1 == true && Sensors_20.O_28_Cart_Stat == true && Sensors_20.O_26_Cart_Stat == false && Sensors_20.O_25_Cart_Stat == false && Sensors_20.O_24_Cart_Stat == false && Sensors_20.O_29_Cart_Stat == false]
    Config_Cv27 -> DeSorting_Cv27 [order 4] : [St_Cv27_1 == true && Sensors_20.O_29_Cart_Stat == true && Sensors_20.O_26_Cart_Stat == false && Sensors_20.O_25_Cart_Stat == false && Sensors_20.O_24_Cart_Stat == false]
  state CartToProcessing3
    state DeRobot_Cv28
      entry:
      St_Cv28_2a = false;
      during:
      % FB11 N2: abre caminho vindo de Robot (27) - prioridade 1
      % ordem do ladder: carro mais proximo a montante do laco
      if Control_20.C_28_Request && Sensors_20.O_27_Cart_Stat
      St_Cv28_2a = true;
      else
      St_Cv28_2a = false;
      end
    state DeVision_Cv28
      entry:
      St_Cv28_2b = false;
      during:
      % FB11 N2: abre caminho vindo de Vision (26) - prioridade 2
      % ordem do ladder: carro mais proximo a montante do laco
      if Control_20.C_28_Request && Sensors_20.O_26_Cart_Stat && ~Sensors_20.O_27_Cart_Stat
      St_Cv28_2b = true;
      else
      St_Cv28_2b = false;
      end
    state Config_Cv28
      entry:
      St_Cv28_1 = false;
      during:
      % FB11 N1: solicitacao de carrinho para Storage
      if Control_20.C_28_Request
      St_Cv28_1 = true;
      else
      St_Cv28_1 = false;
      end
    state EsteiraLigada_Cv28
      entry:
      St_Cv28_3 = false;
      during:
      % FB11 N3: aciona a esteira (exige a controladora ligada)
      if Actuators_20.F_22_Conveyor && Sensors_20.O_20_Controler_On
      St_Cv28_3 = true;
      else
      St_Cv28_3 = false;
      end
    state CarroProximo_Cv28
      entry:
      St_Cv28_4 = false;
      during:
      % FB11 N4: carro proximo da estacao, desliga os pinos
      if Sensors_20.O_28_Cart_Next
      St_Cv28_4 = true;
      else
      St_Cv28_4 = false;
      end
    state IdentificaCarro_Cv28
      entry:
      St_Cv28_5 = false;
      during:
      % FB11 N5: contador identifica o numero do carro
      if Sensors_20.O_28_Count || Sensors_20.O_28_Pist_Bck
      St_Cv28_5 = true;
      else
      St_Cv28_5 = false;
      end
    state CarroChegou_Cv28
      entry:
      St_Cv28_6 = false;
      during:
      % FB11 N6: carro na estacao (T = 3s antes de resetar)
      if Sensors_20.O_28_Cart_Stat && Sensors_20.O_28_Optic
      St_Cv28_6 = true;
      else
      St_Cv28_6 = false;
      end
    state SinalizaChegada_Cv28
      entry:
      St_Cv28_7 = false;
      during:
      % FB11 N7: sinaliza chegada do carro
      if Control_20.C_28_CartDel
      St_Cv28_7 = true;
      else
      St_Cv28_7 = false;
      end
    state DeProcessing_Cv28
      entry:
      St_Cv28_2c = false;
      during:
      % FB11 N2: abre caminho vindo de Processing (25) - prioridade 3
      % ordem do ladder: carro mais proximo a montante do laco
      if Control_20.C_28_Request && Sensors_20.O_25_Cart_Stat && ~Sensors_20.O_27_Cart_Stat && ~Sensors_20.O_26_Cart_Stat
      St_Cv28_2c = true;
      else
      St_Cv28_2c = false;
      end
    state DeTesting_Cv28
      entry:
      St_Cv28_2d = false;
      during:
      % FB11 N2: abre caminho vindo de Testing (24) - prioridade 4
      % ordem do ladder: carro mais proximo a montante do laco
      if Control_20.C_28_Request && Sensors_20.O_24_Cart_Stat && ~Sensors_20.O_27_Cart_Stat && ~Sensors_20.O_26_Cart_Stat && ~Sensors_20.O_25_Cart_Stat
      St_Cv28_2d = true;
      else
      St_Cv28_2d = false;
      end
    state DeSorting_Cv28
      entry:
      St_Cv28_2e = false;
      during:
      % FB11 N2: abre caminho vindo de Sorting (29) - prioridade 5
      % ordem do ladder: carro mais proximo a montante do laco
      if Control_20.C_28_Request && Sensors_20.O_29_Cart_Stat && ~Sensors_20.O_27_Cart_Stat && ~Sensors_20.O_26_Cart_Stat && ~Sensors_20.O_25_Cart_Stat && ~Sensors_20.O_24_Cart_Stat
      St_Cv28_2e = true;
      else
      St_Cv28_2e = false;
      end
    Config_Cv28 -> DeRobot_Cv28 [order 1] : [Control_20.C_28_Request == true && Sensors_20.O_27_Cart_Stat == true]
    DeRobot_Cv28 -> EsteiraLigada_Cv28 : [St_Cv28_2a == true]
    Config_Cv28 -> DeVision_Cv28 [order 2] : [Control_20.C_28_Request == true && Sensors_20.O_26_Cart_Stat == true && Sensors_20.O_27_Cart_Stat == false]
    (default) -> Config_Cv28
    DeVision_Cv28 -> EsteiraLigada_Cv28 : [St_Cv28_2b == true]
    DeProcessing_Cv28 -> EsteiraLigada_Cv28 : [St_Cv28_2c == true]
    DeTesting_Cv28 -> EsteiraLigada_Cv28 : [St_Cv28_2d == true]
    Config_Cv28 -> DeProcessing_Cv28 [order 3] : [Control_20.C_28_Request == true && Sensors_20.O_25_Cart_Stat == true && Sensors_20.O_27_Cart_Stat == false && Sensors_20.O_26_Cart_Stat == false]
    DeSorting_Cv28 -> EsteiraLigada_Cv28 : [St_Cv28_2e == true]
    EsteiraLigada_Cv28 -> CarroProximo_Cv28 : [St_Cv28_3 == true]
    CarroProximo_Cv28 -> IdentificaCarro_Cv28 : [St_Cv28_4 == true]
    IdentificaCarro_Cv28 -> CarroChegou_Cv28 : [St_Cv28_5 == true]
    CarroChegou_Cv28 -> SinalizaChegada_Cv28 : [St_Cv28_6 == true && (Control_20.C_28_CartDel == true || after(3, sec))]
    Config_Cv28 -> DeSorting_Cv28 [order 5] : [Control_20.C_28_Request == true && Sensors_20.O_29_Cart_Stat == true && Sensors_20.O_27_Cart_Stat == false && Sensors_20.O_26_Cart_Stat == false && Sensors_20.O_25_Cart_Stat == false && Sensors_20.O_24_Cart_Stat == false]
    Config_Cv28 -> DeTesting_Cv28 [order 4] : [Control_20.C_28_Request == true && Sensors_20.O_24_Cart_Stat == true && Sensors_20.O_27_Cart_Stat == false && Sensors_20.O_26_Cart_Stat == false && Sensors_20.O_25_Cart_Stat == false]
  state CartToProcessing4
    state DeStorage_Cv29
      entry:
      St_Cv29_2a = false;
      during:
      % FB11 N2: abre caminho vindo de Storage (28) - prioridade 1
      % ordem do ladder: carro mais proximo a montante do laco
      if Control_20.C_29_Request && Sensors_20.O_28_Cart_Stat
      St_Cv29_2a = true;
      else
      St_Cv29_2a = false;
      end
    state DeRobot_Cv29
      entry:
      St_Cv29_2b = false;
      during:
      % FB11 N2: abre caminho vindo de Robot (27) - prioridade 2
      % ordem do ladder: carro mais proximo a montante do laco
      if Control_20.C_29_Request && Sensors_20.O_27_Cart_Stat && ~Sensors_20.O_28_Cart_Stat
      St_Cv29_2b = true;
      else
      St_Cv29_2b = false;
      end
    state Config_Cv29
      entry:
      St_Cv29_1 = false;
      during:
      % FB11 N1: solicitacao de carrinho para Sorting
      if Control_20.C_29_Request
      St_Cv29_1 = true;
      else
      St_Cv29_1 = false;
      end
    state EsteiraLigada_Cv29
      entry:
      St_Cv29_3 = false;
      during:
      % FB11 N3: aciona a esteira (exige a controladora ligada)
      if Actuators_20.F_22_Conveyor && Sensors_20.O_20_Controler_On
      St_Cv29_3 = true;
      else
      St_Cv29_3 = false;
      end
    state CarroProximo_Cv29
      entry:
      St_Cv29_4 = false;
      during:
      % FB11 N4: carro proximo da estacao, desliga os pinos
      if Sensors_20.O_29_Cart_Next
      St_Cv29_4 = true;
      else
      St_Cv29_4 = false;
      end
    state IdentificaCarro_Cv29
      entry:
      St_Cv29_5 = false;
      during:
      % FB11 N5: contador identifica o numero do carro
      if Sensors_20.O_29_Count || Sensors_20.O_29_Pist_Bck
      St_Cv29_5 = true;
      else
      St_Cv29_5 = false;
      end
    state CarroChegou_Cv29
      entry:
      St_Cv29_6 = false;
      during:
      % FB11 N6: carro na estacao (T = 3s antes de resetar)
      if Sensors_20.O_29_Cart_Stat && Sensors_20.O_29_Optic
      St_Cv29_6 = true;
      else
      St_Cv29_6 = false;
      end
    state SinalizaChegada_Cv29
      entry:
      St_Cv29_7 = false;
      during:
      % FB11 N7: sinaliza chegada do carro
      if Control_20.C_29_CartDel
      St_Cv29_7 = true;
      else
      St_Cv29_7 = false;
      end
    state DeVision_Cv29
      entry:
      St_Cv29_2c = false;
      during:
      % FB11 N2: abre caminho vindo de Vision (26) - prioridade 3
      % ordem do ladder: carro mais proximo a montante do laco
      if Control_20.C_29_Request && Sensors_20.O_26_Cart_Stat && ~Sensors_20.O_28_Cart_Stat && ~Sensors_20.O_27_Cart_Stat
      St_Cv29_2c = true;
      else
      St_Cv29_2c = false;
      end
    state DeProcessing_Cv29
      entry:
      St_Cv29_2d = false;
      during:
      % FB11 N2: abre caminho vindo de Processing (25) - prioridade 4
      % ordem do ladder: carro mais proximo a montante do laco
      if Control_20.C_29_Request && Sensors_20.O_25_Cart_Stat && ~Sensors_20.O_28_Cart_Stat && ~Sensors_20.O_27_Cart_Stat && ~Sensors_20.O_26_Cart_Stat
      St_Cv29_2d = true;
      else
      St_Cv29_2d = false;
      end
    state DeTesting_Cv29
      entry:
      St_Cv29_2e = false;
      during:
      % FB11 N2: abre caminho vindo de Testing (24) - prioridade 5
      % ordem do ladder: carro mais proximo a montante do laco
      if Control_20.C_29_Request && Sensors_20.O_24_Cart_Stat && ~Sensors_20.O_28_Cart_Stat && ~Sensors_20.O_27_Cart_Stat && ~Sensors_20.O_26_Cart_Stat && ~Sensors_20.O_25_Cart_Stat
      St_Cv29_2e = true;
      else
      St_Cv29_2e = false;
      end
    Config_Cv29 -> DeStorage_Cv29 [order 1] : [Control_20.C_29_Request == true && Sensors_20.O_28_Cart_Stat == true]
    DeStorage_Cv29 -> EsteiraLigada_Cv29 : [St_Cv29_2a == true]
    Config_Cv29 -> DeRobot_Cv29 [order 2] : [Control_20.C_29_Request == true && Sensors_20.O_27_Cart_Stat == true && Sensors_20.O_28_Cart_Stat == false]
    (default) -> Config_Cv29
    DeRobot_Cv29 -> EsteiraLigada_Cv29 : [St_Cv29_2b == true]
    DeVision_Cv29 -> EsteiraLigada_Cv29 : [St_Cv29_2c == true]
    EsteiraLigada_Cv29 -> CarroProximo_Cv29 : [St_Cv29_3 == true]
    CarroProximo_Cv29 -> IdentificaCarro_Cv29 : [St_Cv29_4 == true]
    IdentificaCarro_Cv29 -> CarroChegou_Cv29 : [St_Cv29_5 == true]
    DeProcessing_Cv29 -> EsteiraLigada_Cv29 : [St_Cv29_2d == true]
    DeTesting_Cv29 -> EsteiraLigada_Cv29 : [St_Cv29_2e == true]
    CarroChegou_Cv29 -> SinalizaChegada_Cv29 : [St_Cv29_6 == true && (Control_20.C_29_CartDel == true || after(3, sec))]
    Config_Cv29 -> DeVision_Cv29 [order 3] : [Control_20.C_29_Request == true && Sensors_20.O_26_Cart_Stat == true && Sensors_20.O_28_Cart_Stat == false && Sensors_20.O_27_Cart_Stat == false]
    Config_Cv29 -> DeProcessing_Cv29 [order 4] : [Control_20.C_29_Request == true && Sensors_20.O_25_Cart_Stat == true && Sensors_20.O_28_Cart_Stat == false && Sensors_20.O_27_Cart_Stat == false && Sensors_20.O_26_Cart_Stat == false]
    Config_Cv29 -> DeTesting_Cv29 [order 5] : [Control_20.C_29_Request == true && Sensors_20.O_24_Cart_Stat == true && Sensors_20.O_28_Cart_Stat == false && Sensors_20.O_27_Cart_Stat == false && Sensors_20.O_26_Cart_Stat == false && Sensors_20.O_25_Cart_Stat == false]
  RBS -> Start : [StatusRBS_5 == true]
  RSB -> Start : [StatusRSB_5 == true]
  (default) -> Start
  BRS -> Start : [StatusBRS_5 == true]
  BSR -> Start : [StatusBSR_5 == true]
  SRB -> Start : [StatusSRB_5 == true]
  Start -> CartToTesting : [Control_20.C_24_Request == true]
  SBR -> Start : [StatusSBR_5 == true]
  (junction 2436) -> BRS : [Control_60.C_65_BRS_Output == true]
  (junction 2433) -> (junction 2436) [order 2]
  CartToTesting -> (junction 1047) : [Control_20.C_24_CartDel == true]
  (junction 1047) -> (junction 1049)
  (junction 2151) -> CartToTesting : [Control_20.C_24_Request == true]
  Handling1_Cart2Del -> (junction 2151) [order 2]
  Distribution_Single -> (junction 829) : [Control_80.C_85_Part_Del == true]
  (junction 832) -> Identified_Delivery
  Identified_Delivery -> (junction 968) : [Control_70.C_75_Part_Del == true]
  (junction 829) -> (junction 826)
  (junction 831) -> (junction 832) [order 2] : [Control_70.C_75_Identified == true]
  (junction 968) -> (junction 971)
  (junction 729) -> (junction 999)
  (junction 999) -> Distribution_Single
  (junction 726) -> (junction 729) [order 1] : [Control_80.C_85_Single == true]
  (junction 993) -> (junction 999) : [Control_70.C_75_RQ_Wrong == true]
  (junction 2433) -> BSR [order 1] : [Control_60.C_65_BSR_Output == true]
  (junction 2430) -> (junction 2433) [order 2]
  (junction 971) -> (junction 1044)
  (junction 1044) -> CartToProcessing : [Control_20.C_25_Request == true]
  (junction 967) -> (junction 971)
  (junction 2430) -> RBS [order 1] : [Control_60.C_65_RBS_Output == true]
  (junction 1049) -> (junction 726)
  (junction 726) -> (junction 996) [order 3] : [Control_80.C_85_Continuous == true]
  (junction 996) -> Distribution_Continuous
  Distribution_Continuous -> (junction 826) : [Control_80.C_85_Part_Del == true]
  (junction 826) -> (junction 831)
  (junction 2420) -> (junction 2430) [order 1]
  (junction 726) -> (junction 732) [order 2] : [Control_80.C_85_Counted == true]
  (junction 992) -> (junction 996) [order 1] : [Control_70.C_75_RQ_Wrong == true]
  (junction 827) -> (junction 826)
  (junction 831) -> (junction 833) [order 1] : [Control_70.C_75_Requested == true]
  Handling1_Cart2Del -> (junction 2420) [order 1] : [Control_50.C_55_PD_Sort == true]
  (junction 2420) -> (junction 2421) [order 2]
  (junction 2143) -> Handling1_Cart2Del
  CartToProcessing4 -> (junction 2143) : [Control_20.C_29_CartDel == true]
  Distribution_Counted -> (junction 827) : [Control_80.C_85_Part_Del == true]
  (junction 732) -> (junction 987)
  (junction 987) -> Distribution_Counted
  (junction 833) -> Requested_Delivery
  Requested_Delivery -> (junction 967) [order 1] : [Control_70.C_75_Part_Del == true]
  (junction 982) -> (junction 987) [order 1] : [Control_70.C_75_RQ_Wrong == true]
  (junction 2141) -> CartToProcessing4 : [Control_20.C_29_Request == true]
  (junction 2140) -> (junction 2141)
  Requested_Delivery -> (junction 965) [order 2] : [Control_70.C_75_RQ_Wrong == true]
  (junction 992) -> (junction 993) [order 2]
  (junction 982) -> (junction 992) [order 2]
  (junction 965) -> (junction 982)
  PartToProcessing -> Processing_TestOnly [order 1] : [Control_90.C_95_PD_Proc == true && Control_100.C_105_Test == true]
  (junction 2421) -> RSB [order 1] : [Control_60.C_65_RSB_Output == true]
  (junction 2061) -> (junction 2140)
  (junction 2421) -> (junction 2424) [order 2]
  (junction 2064) -> Store
  (junction 2060) -> (junction 2064) [order 2] : [Control_40.C_45_StorePart == true]
  (junction 1506) -> PartToProcessing
  CartToProcessing -> (junction 1506) : [Control_20.C_25_CartDel == true]
  Processing_TestOnly -> ProcessingToPart : [Control_100.C_105_Part_ready == true]
  PartToProcessing -> Processing_TestDrill [order 3] : [Control_90.C_95_PD_Proc == true && Control_100.C_105_TestDrill == true]
  Store -> (junction 2061)
  (junction 2071) -> (junction 2061)
  (junction 2077) -> (junction 2060)
  CartToProcessing3 -> (junction 2077) : [Control_20.C_28_CartDel == true]
  (junction 2060) -> (junction 2074) [order 1] : [Control_40.C_45_RetrievePart == true]
  PartToProcessing -> Processing_RotationOnly [order 2] : [Control_90.C_95_PD_Proc == true && Control_100.C_105_Rotation == true]
  Retrieve -> (junction 2071)
  (junction 2424) -> SRB [order 1] : [Control_60.C_65_SRB_Output == true]
  (junction 2424) -> (junction 2427) [order 2]
  (junction 2074) -> Retrieve
  ProcessingToPart -> (junction 1861) : [(St_P2P1_5_10 == true || P2P1_Armed == true) && Control_90.C_95_PD_Cart == true]
  (junction 1861) -> CartToProcessing1 : [Control_20.C_26_Request == true && (St_P2P1_5_10 == true || P2P1_Armed == true)]
  Processing_TestDrill -> ProcessingToPart : [Control_100.C_105_Part_ready == true]
  Processing_RotationOnly -> ProcessingToPart : [Control_100.C_105_Part_ready == true]
  (junction 2427) -> SBR : [Control_60.C_65_SBR_Output == true]
  (junction 2048) -> (junction 2050)
  (junction 2050) -> CartToProcessing3 : [Control_20.C_28_Request == true]
  (junction 2045) -> (junction 2048)
  Vision -> (junction 2015) : [St_Visn_3 == true]
  (junction 2015) -> (junction 2017)
  Robot1 -> (junction 2045) : [Control_30.C_35_Part_Del == true && AS_i_30.A_34_CRoute_Out == true]
  (junction 2043) -> (junction 2045)
  CartToProcessing1 -> Vision : [Control_20.C_26_CartDel == true]
  (junction 2037) -> Robot1 : [AS_i_30.A_34_Cart_Stat == true && Control_30.C_30_Robot1 == true]
  (junction 2035) -> (junction 2037) [order 1]
  CartToProcessing2 -> (junction 2035) : [Control_20.C_27_CartDel == true]
  (junction 2035) -> (junction 2040) [order 2]
  (junction 2017) -> CartToProcessing2 : [St_Visn_3 == true]
  (junction 2040) -> Robot2 : [AS_i_30.A_34_Cart_Stat == true && Control_30.C_30_Robot2 == true]
  Robot2 -> (junction 2043) : [Control_30.C_35_Part_Del == true && AS_i_30.A_34_CRoute_Out == true]
  data: Control_80 input Bus: B_Control_80; Actuators_80 input Bus: B_Actuators_80; Sensors_80 input Bus: B_Sensors_80; AS_i_70 input Bus: B_AS_i_70; Control_70 input Bus: B_Control_70; Actuators_70 input Bus: B_Actuators_70; Sensors_70 input Bus: B_Sensors_70; C_82_Profibus local; C_83_RQ_Parts local; C_85_Continuous local; C_85_Counted local; C_85_Initialization local; C_85_Part_Del local; C_85_Single local; C_85_Start local; F_82_Arm_2_Del local; F_82_Arm_2_Mag local; F_82_Pist_Adv local; F_82_Suction_Off local; F_82_Suction_On local; F_83_Led_Extra1 local; F_83_Led_Extra2 local; F_83_Led_Reset local; F_83_Led_Start local; F_83_Panel_O4 local; F_83_Panel_O5 local; F_83_Panel_O6 local; F_83_Panel_O7 local; O_80_Arm_Del local; O_80_Arm_Mag local; O_80_Mag_Empty local; O_80_Mag_Full local; O_80_Part_Stuck local; O_80_Pist_Back local; O_80_Pist_Fwd local; O_81_Key_Pos local; O_81_Panel_I4 local; O_81_Panel_I5 local; O_81_Panel_I6 local; O_81_Panel_I7 local; O_81_Reset local; O_81_Start local; O_81_Stop local; C_75_ID_Delivery1 local; C_75_ID_Delivery2 local; C_75_Identified local; C_75_Identified80 local; C_75_Initialization local; C_75_Part_Del local; C_75_RQ_Delivery1 local; C_75_RQ_Delivery2 local; C_75_RQ_Part_Del local; C_75_RQ_Wrong local; C_75_Requested local; C_75_Requested80 local; F_72_Air_On local; F_72_Eject_Part local; F_72_Elev_Down local; F_72_Elev_Up local; F_73_Led_Extra1 local; F_73_Led_Extra2 local; F_73_Led_Reset local; F_73_Led_Start local; F_73_Panel_O4 local; F_73_Panel_O5 local; F_73_Panel_O6 local; F_73_Panel_O7 local; O_70_Elev_High local; O_70_Elev_Low local; O_70_Pist_Back local; O_70_SInductive local; O_70_SPart local; O_70_SPart_Height local; O_70_SStation local; O_71_Key_Pos local; O_71_Panel_I4 local; O_71_Panel_I5 local; O_71_Panel_I6 local; O_71_Panel_I7 local; O_71_Reset local; O_71_Start local; O_71_Stop local; A_73_TestCartID local; A_74_CRoute_In local; A_74_CRoute_In80 local; A_74_CRoute_Out local; A_74_Cart_Full local; A_74_Cart_Next local; A_74_Cart_Stat local; A_74_Count local; A_74_No_Cart local; A_74_Optic local; A_74_Pist_Bck local; A_74_Release_FB local; A_74_Request local; C_72_Profibus local; AS_i_30 input Bus: B_AS_i_30; AS_i_50 input Bus: B_AS_i_50; AS_i_90 input Bus: B_AS_i_90; Actuators_100 input Bus: B_Actuators_100; Actuators_20 input Bus: B_Actuators_20; Actuators_30 input Bus: B_Actuators_30; Actuators_50 input Bus: B_Actuators_50; Actuators_60 input Bus: B_Actuators_60; Actuators_90 input Bus: B_Actuators_90; Control_100 input Bus: B_Control_100; Control_20 input Bus: B_Control_20; Control_30 input Bus: B_Control_30; Control_50 input Bus: B_Control_50; Control_60 input Bus: B_Control_60; Control_90 input Bus: B_Control_90; Sensors_100 input Bus: B_Sensors_100; Sensors_20 input Bus: B_Sensors_20; Sensors_30 input Bus: B_Sensors_30; Sensors_50 input Bus: B_Sensors_50; Sensors_60 input Bus: B_Sensors_60; Sensors_90 input Bus: B_Sensors_90; A_32_RoboCartID local; A_34_CRoute_In local; A_34_CRoute_Out local; A_34_Cart_Full local; A_34_Cart_Next local; A_34_Cart_Stat local; A_34_Count local; A_34_No_Cart local; A_34_Optic local; A_34_Pist_Bck local; A_34_Release_FB local; A_34_Request local; A_53_SortCartID local; A_54_CRoute_In local; A_54_CRoute_Out local; A_54_Cart_Full local; A_54_Cart_Next local; A_54_Cart_Stat local; A_54_Count local; A_54_No_Cart local; A_54_Optic local; A_54_Pist_Bck local; A_54_Release_FB local; A_54_Request local; A_93_ProcCartID local; A_94_CRoute_In local; A_94_CRoute_Out local; A_94_Cart_Full local; A_94_Cart_Next local; A_94_Cart_Stat local; A_94_Count local; A_94_No_Cart local; A_94_Optic local; A_94_Pist_Bck local; A_94_Release_FB local; A_94_Request local; C_102_Profibus local; C_103_RQ_Turns local; C_105_Initialization local; C_105_Part_ready local; C_105_Rotation local; C_105_Start local; C_105_Test local; C_105_TestDrill local; C_105_Test_Fail local; C_105_Test_Ok local; C_24_CRoute_In local; C_24_CRoute_Out local; C_24_CartDel local; C_24_Request local; C_25_CRoute_In local; C_25_CRoute_Out local; C_25_CartDel local; C_25_Request local; C_26_CRoute_In local; C_26_CRoute_Out local; C_26_CartDel local; C_26_Request local; C_27_CRoute_In local; C_27_CRoute_Out local; C_27_CartDel local; C_27_Request local; C_28_CRoute_In local; C_28_CRoute_Out local; C_28_CartDel local; C_28_Request local; C_29_CRoute_In local; C_29_CRoute_Out local; C_29_CartDel local; C_29_Request local; C_30_Robot1 local; C_30_Robot2 local; C_35_Part_Del local; C_52_Profibus local; C_55_Cart2Del local; C_55_Initialization local; C_55_PD_Sort local; C_55_Start local; C_62_Profibus local; C_65_BRS_Output local; C_65_BSR_Output local; C_65_ID_1 local; C_65_ID_2 local; C_65_Initialization local; C_65_RBS_Output local; C_65_RSB_Output local; C_65_SBR_Output local; C_65_SRB_Output local; C_92_Profibus local; C_95_Cart2Del local; C_95_Del2Cart local; C_95_Initialization local; C_95_PD_Cart local; C_95_PD_Proc local; C_95_Start local; F_102_Drill_Down local; F_102_Drill_On local; F_102_Drill_Pin local; F_102_Drill_Up local; F_102_RT_On local; F_102_Test_Pin local; F_103_Led_Extra1 local; F_103_Led_Extra2 local; F_103_Led_Reset local; F_103_Led_Start local; F_103_Panel_O4 local; F_103_Panel_O5 local; F_103_Panel_O6 local; F_103_Panel_O7 local; F_22_Led_Off local; F_22_Led_On local; F_24_Release_FB local; F_25_Release_FB local; F_26_Release_FB local; F_27_Release_FB local; F_28_Release_FB local; F_29_Release_FB local; F_33_Cover_Cyl local; F_33_Led_Extra1 local; F_33_Led_Extra2 local; F_33_Led_Reset local; F_33_Led_Start local; F_33_Spring_Cyl local; F_52_Claw_2_Cart local; F_52_Claw_2_Del local; F_52_Claw_Down local; F_52_Close_Claw local; F_53_Led_Extra1 local; F_53_Led_Extra2 local; F_53_Led_Reset local; F_53_Led_Start local; F_53_Panel_O4 local; F_53_Panel_O5 local; F_53_Panel_O6 local; F_53_Panel_O7 local; F_62_Conveyor local; F_62_Identify local; F_62_P1 local; F_62_P2 local; F_63_Led_Extra1 local; F_63_Led_Extra2 local; F_63_Led_Reset local; F_63_Led_Start local; F_63_Panel_O4 local; F_63_Panel_O5 local; F_63_Panel_O6 local; F_63_Panel_O7 local; F_92_Claw_2_Cart local; F_92_Claw_2_Del local; F_92_Claw_Down local; F_92_Close_Claw local; F_93_Led_Extra1 local; F_93_Led_Extra2 local; F_93_Led_Reset local; F_93_Led_Start local; F_93_Panel_O4 local; F_93_Panel_O5 local; F_93_Panel_O6 local; F_93_Panel_O7 local; O_100_PDrill_Pos local; O_100_PInit_Pos local; O_100_PTest_Ok local; O_100_PTest_Pos local; O_100_RT_Sensor local; O_100_SDrill_High local; O_100_SDrill_Low local; O_101_Key_Pos local; O_101_Panel_I4 local; O_101_Panel_I5 local; O_101_Panel_I6 local; O_101_Panel_I7 local; O_101_Reset local; O_101_Start local; O_101_Stop local; O_20_Controler_On local; O_20_Off local; O_20_On local; O_24_Cart_Next local; O_24_Cart_Stat local; O_24_Count local; O_24_Optic local; O_24_Pist_Bck local; O_25_Cart_Next local; O_25_Cart_Stat local; O_25_Count local; O_25_Optic local; O_25_Pist_Back local; O_26_Cart_Next local; O_26_Cart_Stat local; O_26_Count local; O_26_Optic local; O_26_Pist_Back local; O_27_Cart_Next local; O_27_Cart_Stat local; O_27_Count local; O_27_Optic local; O_27_Pist_Back local; O_28_Cart_Next local; O_28_Cart_Stat local; O_28_Count local; O_28_Optic local; O_28_Pist_Back local; O_29_Cart_Next local; O_29_Cart_Stat local; O_29_Count local; O_29_Optic local; O_29_Pist_Back local; O_31_Orientation local; O_31_Part_in_Claw local; O_31_Reset local; O_31_Start local; O_31_Stop local; O_32_CoMag_Empty local; O_32_Co_Cyl_Bck local; O_32_Co_Cyl_Fwd local; O_32_Co_PickUp local; O_32_Sp_Cyl_Bck local; O_32_Sp_Cyl_Fwd local; O_32_Sp_PickUp local; O_50_Claw_Cart local; O_50_Claw_Del local; O_50_Claw_High local; O_50_Claw_Low local; O_50_Claw_Reserve local; O_50_Part_Reserve local; O_50_Part_in_Claw local; O_51_Key_Pos local; O_51_Panel_I4 local; O_51_Panel_I5 local; O_51_Panel_I6 local; O_51_Panel_I7 local; O_51_Reset local; O_51_Start local; O_51_Stop local; O_60_Part_Pass local; O_60_SL1_Bck local; O_60_SL1_Fwd local; O_60_SL2_Bck local; O_60_SL2_Fwd local; O_60_SPart local; O_60_SPhoto local; O_60_Slnd local; O_61_Key_Pos local; O_61_Panel_I4 local; O_61_Panel_I5 local; O_61_Panel_I6 local; O_61_Panel_I7 local; O_61_Reset local; O_61_Start local; O_61_Stop local; O_90_Claw_Cart local; O_90_Claw_Del local; O_90_Claw_High local; O_90_Claw_Low local; O_90_Claw_Reserve local; O_90_Part_Reserve local; O_90_Part_in_Claw local; O_91_Key_Pos local; O_91_Panel_I4 local; O_91_Panel_I5 local; O_91_Panel_I6 local; O_91_Panel_I7 local; O_91_Reset local; O_91_Start local; O_91_Stop local; F_22_Conveyor local; status6 local; status local; status2 local; status3 local; status4 local; status5 local; status7 local; status1 local; status10 local; status11 local; status12 local; status13 local; status9 local; status8 local; status14 local; LoopDistCont local; Control_40 input Bus: B_Control_40; AS_i_40 input Bus: B_AS_i_40; Actuators_40 input Bus: B_Actuators_40; Sensors_40 input Bus: B_Sensors_40; A_44_CRoute_In local; A_44_CRoute_Out local; A_44_Cart_Full local; A_44_Cart_Next local; A_44_Cart_Stat local; A_44_Count local; A_44_No_Cart local; A_44_Optic local; A_44_Pist_Bck local; A_44_Release_FB local; A_44_Request local; C_42_Profibus local; C_45_Initialization local; C_45_RetrievePart local; C_45_Start local; C_45_StorePart local; F_43_Led_Extra1 local; F_43_Led_Extra2 local; F_43_Led_Reset local; F_43_Led_Start local; F_43_Panel_O4 local; F_43_Panel_O5 local; F_43_Panel_O6 local; F_43_Panel_O7 local; O_41_Key_Pos local; O_41_Panel_I4 local; O_41_Panel_I5 local; O_41_Panel_I6 local; O_41_Panel_I7 local; O_41_Reset local; O_41_Start local; O_41_Stop local; C_86_Mag_Parts local; A_43_StorCartID local; C_85_Part_Mag local; C_87_RQ_MParts local; MetalicPart local; Part_Equal local; Part_Different local; status15 local; status16 local; status18 local; status17 local; status19 local; S1_3 local; S1_2 local; S1_1 local; S1_5 local; S1_6 local; S1_4 local; St_DCd0_2c_4 local boolean =false; St_DCd0_2c_1 local boolean =false; St_DCd0_2c_10 local boolean =false; St_DCd0_2c_11 local boolean =false; St_DCd0_2c_12 local boolean =false; St_DCd0_2c_13 local boolean =false; St_DCd0_2c_14 local boolean =false; St_DCd0_2c_15 local boolean =false; St_DCd0_2c_16 local boolean =false; St_DCd0_2c_2 local boolean =false; St_DCd0_2c_3 local boolean =false; St_DCd0_2c_5 local boolean =false; St_DCd0_2c_6 local boolean =false; St_DCd0_2c_7 local boolean =false; St_DCd0_2c_8 local boolean =false; St_DCd0_2c_9 local boolean =false; St_DCt0_2b_1 local boolean =false; St_DCt0_2b_10 local boolean =false; St_DCt0_2b_11 local boolean =false; St_DCt0_2b_12 local boolean =false; St_DCt0_2b_13 local boolean =false; St_DCt0_2b_14 local boolean =false; St_DCt0_2b_15 local boolean =false; St_DCt0_2b_16 local boolean =false; St_DCt0_2b_2 local boolean =false; St_DCt0_2b_3 local boolean =false; St_DCt0_2b_4 local boolean =false; St_DCt0_2b_5 local boolean =false; St_DCt0_2b_6 local boolean =false; St_DCt0_2b_7 local boolean =false; St_DCt0_2b_8 local boolean =false; St_DCt0_2b_9 local boolean =false; St_DSg0_2a_1 local boolean =false; St_DSg0_2a_10 local boolean =false; St_DSg0_2a_11 local boolean =false; St_DSg0_2a_12 local boolean =false; St_DSg0_2a_13 local boolean =false; St_DSg0_2a_14 local boolean =false; St_DSg0_2a_15 local boolean =false; St_DSg0_2a_16 local boolean =false; St_DSg0_2a_2 local boolean =false; St_DSg0_2a_3 local boolean =false; St_DSg0_2a_4 local boolean =false; St_DSg0_2a_5 local boolean =false; St_DSg0_2a_6 local boolean =false; St_DSg0_2a_7 local boolean =false; St_DSg0_2a_8 local boolean =false; St_DSg0_2a_9 local boolean =false; St_IdDl_3a_1 local boolean =false; St_IdDl_3a_13 local boolean =false; St_IdDl_3a_8 local boolean =false; St_P2P0_5_1 local boolean =false; St_P2P0_5_10 local boolean =false; St_P2P0_5_2 local boolean =false; St_P2P0_5_3 local boolean =false; St_P2P0_5_4 local boolean =false; St_P2P0_5_5 local boolean =false; St_P2P0_5_6 local boolean =false; St_P2P0_5_7 local boolean =false; St_P2P0_5_8 local boolean =false; St_P2P0_5_9 local boolean =false; St_P2P1_5_1 local boolean =false; St_P2P1_5_10 local boolean =false; St_P2P1_5_2 local boolean =false; St_P2P1_5_3 local boolean =false; St_P2P1_5_4 local boolean =false; St_P2P1_5_5 local boolean =false; St_P2P1_5_6 local boolean =false; St_P2P1_5_7 local boolean =false; St_P2P1_5_8 local boolean =false; St_P2P1_5_9 local boolean =false; St_ROnly_1 local boolean =false; St_ROnly_2 local boolean =false; St_ROnly_3 local boolean =false; St_ROnly_4 local boolean =false; St_ROnly_5 local boolean =false; St_TDrill_1 local boolean =false; St_TDrill_10 local boolean =false; St_TDrill_11 local boolean =false; St_TDrill_2 local boolean =false; St_TDrill_3 local boolean =false; St_TDrill_4 local boolean =false; St_TDrill_5 local boolean =false; St_TDrill_6 local boolean =false; St_TDrill_7 local boolean =false; St_TDrill_8 local boolean =false; St_TDrill_9 local boolean =false; St_TOnly_1 local boolean =false; St_TOnly_2 local boolean =false; St_TOnly_3 local boolean =false; St_TOnly_4 local boolean =false; St_TOnly_5 local boolean =false; St_TOnly_6 local boolean =false; St_TOnly_7 local boolean =false; St_H1_1 local boolean =false; St_H1_2 local boolean =false; St_H1_3 local boolean =false; St_H1_4 local boolean =false; St_H1_5 local boolean =false; St_H1_6 local boolean =false; St_H1_7 local boolean =false; St_H1_8 local boolean =false; St_H1_9 local boolean =false; St_Retr_1 local boolean =false; St_Retr_2 local boolean =false; St_Retr_3 local boolean =false; St_Retr_4 local boolean =false; St_Retr_5 local boolean =false; St_Stor_1 local boolean =false; St_Stor_2 local boolean =false; St_Stor_3 local boolean =false; St_Stor_4 local boolean =false; St_Stor_5 local boolean =false; Status3a_10 local boolean =false; Status3a_11 local boolean =false; Status3a_12 local boolean =false; Status3a_14 local boolean =false; Status3a_15 local boolean =false; Status3a_2 local boolean =false; Status3a_3 local boolean =false; Status3a_4 local boolean =false; Status3a_5 local boolean =false; Status3a_6 local boolean =false; Status3a_7 local boolean =false; Status3a_9 local boolean =false; Status3b15 local boolean =false; Status3b_1 local boolean =false; Status3b_10 local boolean =false; Status3b_11 local boolean =false; Status3b_12 local boolean =false; Status3b_13 local boolean =false; Status3b_14 local boolean =false; Status3b_15 local boolean =false; Status3b_16 local boolean =false; Status3b_17 local boolean =false; Status3b_18 local boolean =false; Status3b_19 local boolean =false; Status3b_2 local boolean =false; Status3b_20 local boolean =false; Status3b_3 local boolean =false; Status3b_4 local boolean =false; Status3b_5 local boolean =false; Status3b_6 local boolean =false; Status3b_7 local boolean =false; Status3b_8 local boolean =false; Status3b_9 local boolean =false; StatusBRS_1 local boolean =false; StatusBRS_2 local boolean =false; StatusBRS_3 local boolean =false; StatusBRS_4 local boolean =false; StatusBRS_5 local boolean =false; StatusBSR_1 local boolean =false; StatusBSR_2 local boolean =false; StatusBSR_3 local boolean =false; StatusBSR_4 local boolean =false; StatusBSR_5 local boolean =false; StatusRBS_1 local boolean =false; StatusRBS_2 local boolean =false; StatusRBS_3 local boolean =false; StatusRBS_4 local boolean =false; StatusRBS_5 local boolean =false; StatusRSB_1 local boolean =false; StatusRSB_2 local boolean =false; StatusRSB_3 local boolean =false; StatusRSB_4 local boolean =false; StatusRSB_5 local boolean =false; StatusSBR_1 local boolean =false; StatusSBR_2 local boolean =false; StatusSBR_3 local boolean =false; StatusSBR_4 local boolean =false; StatusSBR_5 local boolean =false; StatusSRB_1 local boolean =false; StatusSRB_2 local boolean =false; StatusSRB_3 local boolean =false; StatusSRB_4 local boolean =false; StatusSRB_5 local boolean =false; St_Rbt1_1 local boolean =false; St_Rbt1_2 local boolean =false; St_Rbt1_3 local boolean =false; St_Rbt1_4 local boolean =false; St_Rbt1_5 local boolean =false; St_Rbt1_6 local boolean =false; St_Rbt1_7 local boolean =false; St_Rbt2_1 local boolean =false; St_Rbt2_2 local boolean =false; St_Rbt2_3 local boolean =false; St_Rbt2_4 local boolean =false; St_Rbt2_5 local boolean =false; St_Rbt2_6 local boolean =false; St_Rbt2_7 local boolean =false; St_Cv24_1 local boolean =false; St_Cv24_3 local boolean =false; St_Cv24_4 local boolean =false; St_Cv24_5 local boolean =false; St_Cv24_6 local boolean =false; St_Cv24_7 local boolean =false; St_Cv25_1 local boolean =false; St_Cv25_3 local boolean =false; St_Cv25_4 local boolean =false; St_Cv25_5 local boolean =false; St_Cv25_6 local boolean =false; St_Cv25_7 local boolean =false; St_Cv26_1 local boolean =false; St_Cv26_3 local boolean =false; St_Cv26_4 local boolean =false; St_Cv26_5 local boolean =false; St_Cv26_6 local boolean =false; St_Cv26_7 local boolean =false; St_Cv27_1 local boolean =false; St_Cv27_3 local boolean =false; St_Cv27_4 local boolean =false; St_Cv27_5 local boolean =false; St_Cv27_6 local boolean =false; St_Cv27_7 local boolean =false; St_Cv28_1 local boolean =false; St_Cv28_3 local boolean =false; St_Cv28_4 local boolean =false; St_Cv28_5 local boolean =false; St_Cv28_6 local boolean =false; St_Cv28_7 local boolean =false; St_Cv29_1 local boolean =false; St_Cv29_3 local boolean =false; St_Cv29_4 local boolean =false; St_Cv29_5 local boolean =false; St_Cv29_6 local boolean =false; St_Cv29_7 local boolean =false; St_Visn_1 local boolean =false; St_Visn_2 local boolean =false; St_Visn_3 local boolean =false; St_Cv24_2a local boolean =false; St_Cv24_2b local boolean =false; St_Cv24_2c local boolean =false; St_Cv24_2d local boolean =false; St_Cv24_2e local boolean =false; St_Cv25_2a local boolean =false; St_Cv25_2b local boolean =false; St_Cv25_2c local boolean =false; St_Cv25_2d local boolean =false; St_Cv25_2e local boolean =false; St_Cv26_2a local boolean =false; St_Cv26_2b local boolean =false; St_Cv26_2c local boolean =false; St_Cv26_2d local boolean =false; St_Cv26_2e local boolean =false; St_Cv27_2a local boolean =false; St_Cv27_2b local boolean =false; St_Cv27_2c local boolean =false; St_Cv27_2d local boolean =false; St_Cv27_2e local boolean =false; St_Cv28_2a local boolean =false; St_Cv28_2b local boolean =false; St_Cv28_2c local boolean =false; St_Cv28_2d local boolean =false; St_Cv28_2e local boolean =false; St_Cv29_2a local boolean =false; St_Cv29_2b local boolean =false; St_Cv29_2c local boolean =false; St_Cv29_2d local boolean =false; St_Cv29_2e local boolean =false; P2P1_Armed local boolean =false; Vis_Req27 local boolean =false; Vis_RIn local boolean =false; Vis_ROut local boolean =false; Vis_Cart local boolean =false
